simulink model "s_c_nbe_m1k"  (R2016b)
settings: Solver=VariableStepAuto  StartTime=0.0  StopTime=1000  RelTol=1e-3  EnableMultiTasking=on
undefined symbols (not defined in the file): Coeffs, fft_stages, n_taps, output_bits, pfb_coeff_gen_calc, xengbits
libraries: xbsIndex_r4 x23639, casper_library_misc x65, casper_library_scopes x4, xbsReplacements_r4 x4, xps_library x3
(part 19 of 198)

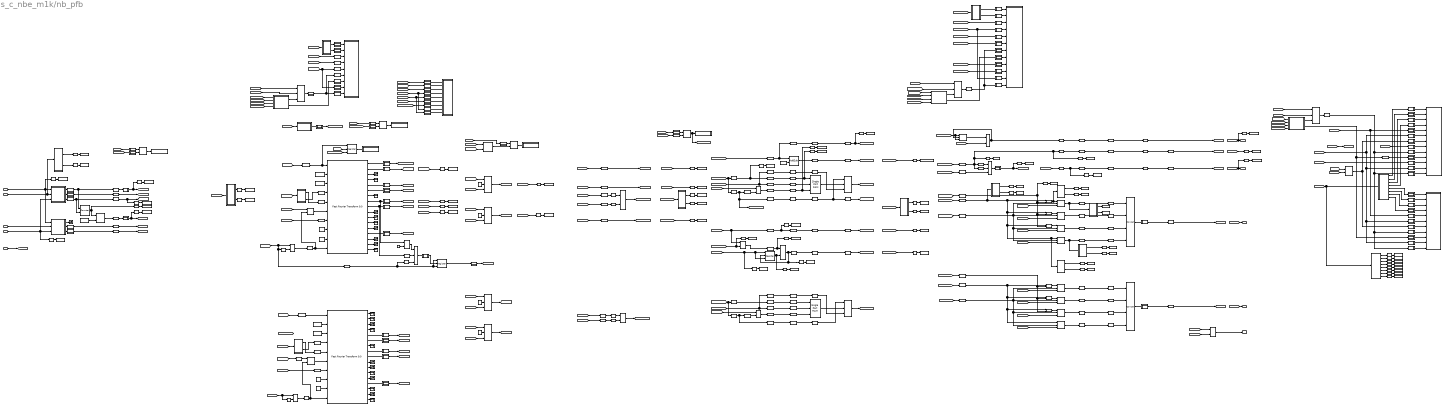
== system s_c_nbe_m1k/nb_pfb ==
  note: FWD = 1
  note: NOTE: Init script Disabled due to change to manual change to sync_delay block
  note: NOTE: The sync must be inline with the DV at this point
  note: Trigger sync on falling edge
  note: NOT ensures that a sync occuring atthe same time as ch=0 will prevent
      | sync from latching the register. The next cycle when sync in =0 the relational check
      | will equal 1  as the input will be zero as the FFT block would have just finished a reset.
  note: Only allow sync to occur when ch=0 and dv=1.
  note: Delay=2 as rst is 2 cycles. Prevents sync from popping out early
  note: Pass sync when first 4 samples have been captured
  note: Sanity check for channel number out
  note: Trigger when half the channels have been written
  note: Check if pol0 and pol1 ch outputs drift.
      | This should never happen.
  note: Needs to be 10b for 1k
  note: Count how many times the current_channel
      | is equal to 2^fft_stages BEFORE the sync occurs.
      | This is needed to compute the new time for the time gen
      | block which follows.
  note: There is no offset of the sync by 3 cycles. This is due to the 1:4
      | sample ratio casued by the capture_now. We want the sync to
      | occur one cycle before DV
  note: Wait for capture_now to trigger after sync has arrived
  note: Trigger capture_now every '4' samples.
      | This is based on the current channel index.
      | This starts at 0, so trigger when current channels
      | lower two bits = '1' and '1' (i.e. decimal 3).
  note: Needs to be 10b for 1k
  note: Trigger when half the channels have been written
  note: NOTE: The sync must be inline with the DV at this point
  note: FWD = 1
  sync : Inport
  pol0 : Inport  Port=2
  pol1 : Inport  Port=3
  dvalid : Inport  Port=4
  fft_shift : Inport  Port=5
  AddSub : xbsIndex_r4/AddSub  mode=Subtraction  use_carryin=off  use_carryout=off  en=off  latency=1  precision=User Defined  arith_type=Unsigned  n_bits=fft_stages-1  bin_pt=0  quantization=Truncate  overflow=Wrap  use_behavioral_HDL=off  hw_selection=Fabric  pipelined=off  dbl_ovrd=off  block_type=addsub
  Concat : xbsIndex_r4/Concat  num_inputs=2  dbl_ovrd=off  block_type=concat
  Concat1 : xbsIndex_r4/Concat  num_inputs=4  dbl_ovrd=off  block_type=concat
  Concat2 : xbsIndex_r4/Concat  num_inputs=2  dbl_ovrd=off  block_type=concat
  Concat3 : xbsIndex_r4/Concat  num_inputs=2  dbl_ovrd=off  block_type=concat
  Concat5 : xbsIndex_r4/Concat  num_inputs=4  dbl_ovrd=off  block_type=concat
  Constant : xbsIndex_r4/Constant  const=0  gui_display_data_type=Fixed-point  arith_type=Unsigned  n_bits=10  bin_pt=0  preci_type=Single  exp_width=8  frac_width=24  explicit_period=on  period=1  equ=P=C  opselect=C  inp2=PCIN>>17  opr=+  inp1=P  carry=CIN  dbl_ovrd=off  block_type=constant
  Constant{1..2,6..7} (4 alike) : xbsIndex_r4/Constant  const=0  gui_display_data_type=Fixed-point  arith_type=Signed (2's comp)  n_bits=18  bin_pt=17  preci_type=Single  exp_width=8  frac_width=24  explicit_period=on  period=1  equ=P=C  opselect=C  inp2=PCIN>>17  opr=+  inp1=P  carry=CIN  dbl_ovrd=off  block_type=constant
  Constant10 : xbsIndex_r4/Constant  const=1  gui_display_data_type=Boolean  arith_type=Boolean  n_bits=1  bin_pt=0  preci_type=Single  exp_width=8  frac_width=24  explicit_period=on  period=1  equ=P=C  opselect=C  inp2=PCIN>>17  opr=+  inp1=P  carry=CIN  dbl_ovrd=off  block_type=constant
  Constant{4,8,11..12} (4 alike) : xbsIndex_r4/Constant  const=1  gui_display_data_type=Boolean  arith_type=Boolean  n_bits=18  bin_pt=17  preci_type=Single  exp_width=8  frac_width=24  explicit_period=on  period=1  equ=P=C  opselect=C  inp2=PCIN>>17  opr=+  inp1=P  carry=CIN  dbl_ovrd=off  block_type=constant
  Constant13 : xbsIndex_r4/Constant  const=1  gui_display_data_type=Boolean  arith_type=Boolean  n_bits=1  bin_pt=0  preci_type=Single  exp_width=8  frac_width=24  explicit_period=on  period=1  equ=P=C  opselect=C  inp2=PCIN>>17  opr=+  inp1=P  carry=CIN  dbl_ovrd=off  block_type=constant
  Constant17 : xbsIndex_r4/Constant  const=2^(fft_stages-2)  gui_display_data_type=Fixed-point  arith_type=Unsigned  n_bits=fft_stages-1  bin_pt=0  preci_type=Single  exp_width=8  frac_width=24  explicit_period=on  period=1  equ=P=C  opselect=C  inp2=PCIN>>17  opr=+  inp1=P  carry=CIN  dbl_ovrd=off  block_type=constant
  Constant3 : xbsIndex_r4/Constant  const=1  gui_display_data_type=Fixed-point  arith_type=Unsigned  n_bits=1  bin_pt=0  preci_type=Single  exp_width=8  frac_width=24  explicit_period=on  period=1  equ=P=C  opselect=C  inp2=PCIN>>17  opr=+  inp1=P  carry=CIN  dbl_ovrd=off  block_type=constant
  Constant5 : xbsIndex_r4/Constant  const=1  gui_display_data_type=Fixed-point  arith_type=Unsigned  n_bits=1  bin_pt=0  preci_type=Single  exp_width=8  frac_width=24  explicit_period=on  period=1  equ=P=C  opselect=C  inp2=PCIN>>17  opr=+  inp1=P  carry=CIN  dbl_ovrd=off  block_type=constant
  Constant9 : xbsIndex_r4/Constant  const=(2^(fft_stages-1))-1  gui_display_data_type=Fixed-point  arith_type=Unsigned  n_bits=fft_stages+1  bin_pt=0  preci_type=Single  exp_width=8  frac_width=24  explicit_period=on  period=1  equ=P=C  opselect=C  inp2=PCIN>>17  opr=+  inp1=P  carry=CIN  dbl_ovrd=off  block_type=constant
  Counter1 : xbsIndex_r4/Counter  cnt_type=Free Running  cnt_to=Inf  operation=Up  start_count=0  cnt_by_val=1  arith_type=Unsigned  n_bits=4  bin_pt=0  load_pin=off  rst=on  en=on  explicit_period=on  period=1  use_behavioral_HDL=off  implementation=DSP48  dbl_ovrd=off  block_type=counter
  Counter12 : xbsIndex_r4/Counter  cnt_type=Free Running  cnt_to=Inf  operation=Up  start_count=0  cnt_by_val=1  arith_type=Unsigned  n_bits=32  bin_pt=0  load_pin=off  rst=on  en=on  explicit_period=on  period=1  use_behavioral_HDL=off  implementation=DSP48  dbl_ovrd=off  block_type=counter
      settings: block_version=11.4
  Counter2 : xbsIndex_r4/Counter  cnt_type=Free Running  cnt_to=Inf  operation=Up  start_count=0  cnt_by_val=1  arith_type=Unsigned  n_bits=32  bin_pt=0  load_pin=off  rst=on  en=on  explicit_period=on  period=1  use_behavioral_HDL=off  implementation=DSP48  dbl_ovrd=off  block_type=counter
      settings: block_version=11.4
  Counter3 : xbsIndex_r4/Counter  cnt_type=Free Running  cnt_to=Inf  operation=Up  start_count=0  cnt_by_val=1  arith_type=Unsigned  n_bits=fft_stages-1  bin_pt=0  load_pin=off  rst=on  en=on  explicit_period=on  period=1  use_behavioral_HDL=off  implementation=Fabric  dbl_ovrd=off  block_type=counter
  Counter4 : xbsIndex_r4/Counter  cnt_type=Free Running  cnt_to=Inf  operation=Up  start_count=0  cnt_by_val=1  arith_type=Unsigned  n_bits=11  bin_pt=0  load_pin=off  rst=on  en=on  explicit_period=on  period=1  use_behavioral_HDL=off  implementation=DSP48  dbl_ovrd=off  block_type=counter
      settings: block_version=11.4
  Counter5 : xbsIndex_r4/Counter  cnt_type=Free Running  cnt_to=Inf  operation=Up  start_count=0  cnt_by_val=1  arith_type=Unsigned  n_bits=8  bin_pt=0  load_pin=off  rst=on  en=on  explicit_period=on  period=1  use_behavioral_HDL=off  implementation=DSP48  dbl_ovrd=off  block_type=counter
      settings: block_version=11.4
  Delay{1..6,8..13,15,17..18,21..35,37..38,41..50,53..63,65,68,73..76,78,86..96,99..117} (90 alike) : xbsIndex_r4/Delay  rst=off  infoeditControl=Selection of Reset will increase slice count due to use of real FFs and instead of SRLs  en=off  latency=1  reg_retiming=off  dbl_ovrd=off  block_type=delay
      settings: infoedit=Hardware notes: A delay line is a chain, each link of which is an SRL16 or SRL32 followed by a flip-flop.
  Delay{14,39..40,67,69..70,81..84,118} (11 alike) : xbsIndex_r4/Delay  rst=off  infoeditControl=Selection of Reset will increase slice count due to use of real FFs and instead of SRLs  en=off  latency=2  reg_retiming=off  dbl_ovrd=off  block_type=delay
      settings: infoedit=Hardware notes: A delay line is a chain, each link of which is an SRL16 or SRL32 followed by a flip-flop.
  Delay16 : xbsIndex_r4/Delay  rst=off  infoeditControl=Selection of Reset will increase slice count due to use of real FFs and instead of SRLs  en=on  latency=3  reg_retiming=off  dbl_ovrd=off  block_type=delay
      settings: infoedit=Hardware notes: A delay line is a chain, each link of which is an SRL16 or SRL32 followed by a flip-flop.
  Delay19 : xbsIndex_r4/Delay  rst=off  infoeditControl=Selection of Reset will increase slice count due to use of real FFs and instead of SRLs  en=on  latency=2  reg_retiming=off  dbl_ovrd=off  block_type=delay
      settings: infoedit=Hardware notes: A delay line is a chain, each link of which is an SRL16 or SRL32 followed by a flip-flop.
  Delay20 : xbsIndex_r4/Delay  rst=off  infoeditControl=Selection of Reset will increase slice count due to use of real FFs and instead of SRLs  en=on  latency=1  reg_retiming=off  dbl_ovrd=off  block_type=delay
      settings: infoedit=Hardware notes: A delay line is a chain, each link of which is an SRL16 or SRL32 followed by a flip-flop.
  Delay51 : xbsIndex_r4/Delay  rst=off  infoeditControl=Selection of Reset will increase slice count due to use of real FFs and instead of SRLs  en=on  latency=2  reg_retiming=off  dbl_ovrd=off  block_type=delay
      settings: infoedit=Hardware notes: A delay line is a chain, each link of which is an SRL16 or SRL32 followed by a flip-flop.
  Delay52 : xbsIndex_r4/Delay  rst=off  infoeditControl=Selection of Reset will increase slice count due to use of real FFs and instead of SRLs  en=on  latency=1  reg_retiming=off  dbl_ovrd=off  block_type=delay
      settings: infoedit=Hardware notes: A delay line is a chain, each link of which is an SRL16 or SRL32 followed by a flip-flop.
  Delay7 : xbsIndex_r4/Delay  rst=off  infoeditControl=Selection of Reset will increase slice count due to use of real FFs and instead of SRLs  en=on  latency=3  reg_retiming=off  dbl_ovrd=off  block_type=delay
      settings: infoedit=Hardware notes: A delay line is a chain, each link of which is an SRL16 or SRL32 followed by a flip-flop.
  Delay97 : xbsIndex_r4/Delay  rst=off  infoeditControl=Selection of Reset will increase slice count due to use of real FFs and instead of SRLs  en=off  latency=1  reg_retiming=on  dbl_ovrd=off  block_type=delay
  Delay98 : xbsIndex_r4/Delay  rst=off  infoeditControl=Selection of Reset will increase slice count due to use of real FFs and instead of SRLs  en=off  latency=1  reg_retiming=on  dbl_ovrd=off  block_type=delay
  Fast Fourier Transform 9.0 1 : xbsIndex_r4/Fast Fourier Transform 9.0   transform_length=1024  target_clock_frequency=240  target_data_throughput=50  implementation_options=pipelined_streaming_io  run_time_configurable_transform_length=off  phase_factor_width=18  scaling_options=scaled  rounding_modes=convergent_rounding  aclken=off  aresetn=on  output_ordering=natural_order  cyclic_prefix_insertion=off  throttle_scheme=nonrealtime  xk_index=on  ovflo=on  trim_axipin_name=on  memory_options_data=block_ram  memory_options_phase_factors=block_ram  number_of_stages_using_block_ram_for_data_and_phase_factors=5  memory_options_reorder=block_ram  memory_options_hybrid=off  complex_mult_type=use_mults_performance  butterfly_type=use_xtremedsp_slices  simulation_type=hybrid_sim  simulation_model=sysgen:xfftv9_cmodel  data_path_portlist={ 's_axis_data_tdata', 'm_axis_data_tdata', 'm_axis_status_tdata', 'event_fft_overflow' }  channels=1  input_ordering=natural_order  input_width=16  ip_name=Fast Fourier Transform  ip_version=9.0  dsptool_ready=true  ipcore_usecache=true  ipcore_useipmodelcache=true  wrapper_available=true  port_translation_map={ 'aclken' => 'en', 'aresetn' => 'rst'}  data_format=fixed_point  block_type=xfft_v9_0
  Fast Fourier Transform 9.0 2 : xbsIndex_r4/Fast Fourier Transform 9.0   transform_length=1024  target_clock_frequency=240  target_data_throughput=50  implementation_options=pipelined_streaming_io  run_time_configurable_transform_length=off  phase_factor_width=18  scaling_options=scaled  rounding_modes=convergent_rounding  aclken=off  aresetn=on  output_ordering=natural_order  cyclic_prefix_insertion=off  throttle_scheme=nonrealtime  xk_index=on  ovflo=on  trim_axipin_name=on  memory_options_data=block_ram  memory_options_phase_factors=block_ram  number_of_stages_using_block_ram_for_data_and_phase_factors=5  memory_options_reorder=block_ram  memory_options_hybrid=off  complex_mult_type=use_mults_performance  butterfly_type=use_xtremedsp_slices  simulation_type=hybrid_sim  simulation_model=sysgen:xfftv9_cmodel  data_path_portlist={ 's_axis_data_tdata', 'm_axis_data_tdata', 'm_axis_status_tdata', 'event_fft_overflow' }  channels=1  input_ordering=natural_order  input_width=16  ip_name=Fast Fourier Transform  ip_version=9.0  dsptool_ready=true  ipcore_usecache=true  ipcore_useipmodelcache=true  wrapper_available=true  port_translation_map={ 'aclken' => 'en', 'aresetn' => 'rst'}  data_format=fixed_point  block_type=xfft_v9_0
  Gateway Out{1..9,11..31,33..40,43,46..53,55..58,61,65..67,70..73,83} (60 alike) : xbsIndex_r4/Gateway Out  inherit_from_input=off  hdl_port=on  rows=1  columns=1  UseAsDAC=off  DACChannel='1'  interface=None  automatic_assignment=on  address_offset=hex2dec('00')  intf_name=''  intf_description=''  timing_constraint=None  locs_specified=off  LOCs={}  io_standard={}  block_type=gatewayout
  Inverter{,1..4} (5 alike) : xbsIndex_r4/Inverter  en=off  latency=0  dbl_ovrd=off  block_type=inv
  Logical : xbsIndex_r4/Logical  logical_function=AND  inputs=3  en=off  latency=0  precision=Full  arith_type=Unsigned  n_bits=16  bin_pt=0  align_bp=on  dbl_ovrd=off  block_type=logical
  Logical{1..3,5..6,8,10} (7 alike) : xbsIndex_r4/Logical  logical_function=AND  inputs=2  en=off  latency=0  precision=Full  arith_type=Unsigned  n_bits=16  bin_pt=0  align_bp=on  dbl_ovrd=off  block_type=logical
  Logical11 : xbsIndex_r4/Logical  logical_function=OR  inputs=2  en=off  latency=0  precision=Full  arith_type=Unsigned  n_bits=16  bin_pt=0  align_bp=on  dbl_ovrd=off  block_type=logical
  Logical4 : xbsIndex_r4/Logical  logical_function=AND  inputs=3  en=off  latency=0  precision=Full  arith_type=Unsigned  n_bits=16  bin_pt=0  align_bp=on  dbl_ovrd=off  block_type=logical
  Logical7 : xbsIndex_r4/Logical  logical_function=OR  inputs=2  en=off  latency=0  precision=Full  arith_type=Unsigned  n_bits=16  bin_pt=0  align_bp=on  dbl_ovrd=off  block_type=logical
  Mux1 : xbsIndex_r4/Mux  inputs=2  en=off  latency=1  precision=Full  arith_type=Unsigned  n_bits=16  bin_pt=14  quantization=Truncate  overflow=Wrap  dbl_ovrd=off  block_type=mux
  Mux{3..6,8..10} (7 alike) : xbsIndex_r4/Mux  inputs=2  en=off  latency=0  precision=Full  arith_type=Unsigned  n_bits=16  bin_pt=14  quantization=Truncate  overflow=Wrap  dbl_ovrd=off  block_type=mux
  Mux11 : xbsIndex_r4/Mux  inputs=2  en=off  latency=1  precision=Full  arith_type=Unsigned  n_bits=16  bin_pt=14  quantization=Truncate  overflow=Wrap  dbl_ovrd=off  block_type=mux
  Register{,1..7,9..12} (12 alike) : xbsIndex_r4/Register  init=0  rst=on  en=on  dbl_ovrd=off  block_type=register
  Reinterpret{,1..3} (4 alike) : xbsIndex_r4/Reinterpret  force_arith_type=on  arith_type=Unsigned  force_bin_pt=on  bin_pt=0  block_type=reinterpret
  Relational1 : xbsIndex_r4/Relational  mode=a!=b  op_type=Bool  en=off  latency=4  dbl_ovrd=off  block_type=relational
  Relational2 : xbsIndex_r4/Relational  mode=a=b  op_type=Bool  en=off  latency=1  dbl_ovrd=off  block_type=relational
  Relational4 : xbsIndex_r4/Relational  mode=a=b  op_type=Bool  en=off  latency=1  dbl_ovrd=off  block_type=relational
  Single Port RAM : xbsIndex_r4/Single Port RAM  depth=2^(fft_stages-2)  initVector=0  distributed_mem=Block RAM  write_mode=Read Before Write  rst=off  init_reg=0  en=off  latency=1  optimize=Area  dbl_ovrd=off  block_type=spram
  Single Port RAM1 : xbsIndex_r4/Single Port RAM  depth=2^(fft_stages-2)  initVector=0  distributed_mem=Block RAM  write_mode=Read Before Write  rst=off  init_reg=0  en=off  latency=1  optimize=Area  dbl_ovrd=off  block_type=spram
  Slice : xbsIndex_r4/Slice  nbits=10  boolean_output=off  mode=Lower Bit Location + Width  bit1=0  base1=MSB of Input  bit0=0  base0=LSB of Input  dbl_ovrd=off  block_type=slice
  Slice1 : xbsIndex_r4/Slice  nbits=10  boolean_output=off  mode=Lower Bit Location + Width  bit1=0  base1=MSB of Input  bit0=0  base0=LSB of Input  dbl_ovrd=off  block_type=slice
  Slice2 : xbsIndex_r4/Slice  nbits=1  boolean_output=on  mode=Lower Bit Location + Width  bit1=0  base1=MSB of Input  bit0=fft_stages-2  base0=LSB of Input  dbl_ovrd=off  block_type=slice
  Slice3 : xbsIndex_r4/Slice  nbits=1  boolean_output=on  mode=Lower Bit Location + Width  bit1=0  base1=MSB of Input  bit0=fft_stages-2  base0=LSB of Input  dbl_ovrd=off  block_type=slice
  Slice4 : xbsIndex_r4/Slice  nbits=fft_stages-2  boolean_output=off  mode=Lower Bit Location + Width  bit1=0  base1=MSB of Input  bit0=0  base0=LSB of Input  dbl_ovrd=off  block_type=slice
  Slice5 : xbsIndex_r4/Slice  nbits=38  boolean_output=off  mode=Lower Bit Location + Width  bit1=0  base1=MSB of Input  bit0=0  base0=LSB of Input  dbl_ovrd=off  block_type=slice
  Slice6 : xbsIndex_r4/Slice  nbits=fft_stages-2  boolean_output=off  mode=Lower Bit Location + Width  bit1=0  base1=MSB of Input  bit0=0  base0=LSB of Input  dbl_ovrd=off  block_type=slice
  Terminator{1..5,7..24} (23 alike) : Terminator
  To Workspace1 : ToWorkspace  VariableName=fir_dv  SaveFormat=Timeseries  SampleTime=-1
  To Workspace11 : ToWorkspace  VariableName=fft_ch_out1  SaveFormat=Timeseries  SampleTime=-1
  To Workspace12 : ToWorkspace  VariableName=cap_tp6  SaveFormat=Timeseries  SampleTime=-1
  To Workspace13 : ToWorkspace  VariableName=cap_tp7  SaveFormat=Timeseries  SampleTime=-1
  To Workspace14 : ToWorkspace  VariableName=cap_tp8  SaveFormat=Timeseries  SampleTime=-1
  To Workspace15 : ToWorkspace  VariableName=fft_re1  SaveFormat=Timeseries  SampleTime=-1
  To Workspace16 : ToWorkspace  VariableName=fft_sync  SaveFormat=Timeseries  SampleTime=-1
  To Workspace17 : ToWorkspace  VariableName=fft_im1  SaveFormat=Timeseries  SampleTime=-1
  To Workspace18 : ToWorkspace  VariableName=fft_tp1  SaveFormat=Timeseries  SampleTime=-1
  To Workspace19 : ToWorkspace  VariableName=nb_dv  SaveFormat=Timeseries  SampleTime=-1
  To Workspace2 : ToWorkspace  VariableName=fft_re  SaveFormat=Timeseries  SampleTime=-1
  To Workspace20 : ToWorkspace  VariableName=fft_tp  SaveFormat=Timeseries  SampleTime=-1
  To Workspace21 : ToWorkspace  VariableName=nb_r0  SaveFormat=Timeseries  SampleTime=-1
  To Workspace22 : ToWorkspace  VariableName=cap_tp21  SaveFormat=Timeseries  SampleTime=-1
  To Workspace23 : ToWorkspace  VariableName=nb_i0  SaveFormat=Timeseries  SampleTime=-1
  To Workspace24 : ToWorkspace  VariableName=nb_r1  SaveFormat=Timeseries  SampleTime=-1
  To Workspace25 : ToWorkspace  VariableName=nb_r2  SaveFormat=Timeseries  SampleTime=-1
  To Workspace26 : ToWorkspace  VariableName=nb_r3  SaveFormat=Timeseries  SampleTime=-1
  To Workspace27 : ToWorkspace  VariableName=nb_i1  SaveFormat=Timeseries  SampleTime=-1
  To Workspace28 : ToWorkspace  VariableName=nb_i2  SaveFormat=Timeseries  SampleTime=-1
  To Workspace29 : ToWorkspace  VariableName=nb_i3  SaveFormat=Timeseries  SampleTime=-1
  To Workspace3 : ToWorkspace  VariableName=fft_dvalid  SaveFormat=Timeseries  SampleTime=-1
  To Workspace30 : ToWorkspace  VariableName=cap_tp22  SaveFormat=Timeseries  SampleTime=-1
  To Workspace31 : ToWorkspace  VariableName=fft_tp2  SaveFormat=Timeseries  SampleTime=-1
  To Workspace32 : ToWorkspace  VariableName=fft_ch  SaveFormat=Timeseries  SampleTime=-1
  To Workspace34 : ToWorkspace  VariableName=fft_tp3  SaveFormat=Timeseries  SampleTime=-1
  To Workspace35 : ToWorkspace  VariableName=fir_p1  SaveFormat=Timeseries  SampleTime=-1
  To Workspace36 : ToWorkspace  VariableName=fir_dv1  SaveFormat=Timeseries  SampleTime=-1
  To Workspace37 : ToWorkspace  VariableName=fft_sync0  SaveFormat=Timeseries  SampleTime=-1
  To Workspace38 : ToWorkspace  VariableName=cap_tp23  SaveFormat=Timeseries  SampleTime=-1
  To Workspace39 : ToWorkspace  VariableName=fir_p  SaveFormat=Timeseries  SampleTime=-1
  To Workspace4 : ToWorkspace  VariableName=fir_re  SaveFormat=Timeseries  SampleTime=-1
  To Workspace40 : ToWorkspace  VariableName=capture_now  SaveFormat=Timeseries  SampleTime=-1
  To Workspace42 : ToWorkspace  VariableName=reord_sync  SaveFormat=Timeseries  SampleTime=-1
  To Workspace43 : ToWorkspace  VariableName=fft_tp4  SaveFormat=Timeseries  SampleTime=-1
  To Workspace45 : ToWorkspace  VariableName=cap_tp9  SaveFormat=Timeseries  SampleTime=-1
  To Workspace46 : ToWorkspace  VariableName=cap_tp10  SaveFormat=Timeseries  SampleTime=-1
  To Workspace47 : ToWorkspace  VariableName=reord_dv  SaveFormat=Timeseries  SampleTime=-1
  To Workspace48 : ToWorkspace  VariableName=fft_tp5  SaveFormat=Timeseries  SampleTime=-1
  To Workspace49 : ToWorkspace  VariableName=nb_dv1  SaveFormat=Timeseries  SampleTime=-1
  To Workspace5 : ToWorkspace  VariableName=fft_im  SaveFormat=Timeseries  SampleTime=-1
  To Workspace51 : ToWorkspace  VariableName=reord_ch  SaveFormat=Timeseries  SampleTime=-1
  To Workspace53 : ToWorkspace  VariableName=fir_tlast  SaveFormat=Timeseries  SampleTime=-1
  To Workspace54 : ToWorkspace  VariableName=fir_tlast1  SaveFormat=Timeseries  SampleTime=-1
  To Workspace56 : ToWorkspace  VariableName=fft_tp6  SaveFormat=Timeseries  SampleTime=-1
  To Workspace57 : ToWorkspace  VariableName=fft_tp7  SaveFormat=Timeseries  SampleTime=-1
  To Workspace58 : ToWorkspace  VariableName=fft_ch_reord  SaveFormat=Timeseries  SampleTime=-1
  To Workspace59 : ToWorkspace  VariableName=fft_tp8  SaveFormat=Timeseries  SampleTime=-1
  To Workspace6 : ToWorkspace  VariableName=fir_sync  SaveFormat=Timeseries  SampleTime=-1
  To Workspace64 : ToWorkspace  VariableName=cap_tp11  SaveFormat=Timeseries  SampleTime=-1
  To Workspace65 : ToWorkspace  VariableName=fft_ch0  SaveFormat=Timeseries  SampleTime=-1
  To Workspace66 : ToWorkspace  VariableName=fft_dv0  SaveFormat=Timeseries  SampleTime=-1
  To Workspace69 : ToWorkspace  VariableName=fft_re2  SaveFormat=Timeseries  SampleTime=-1
  To Workspace7 : ToWorkspace  VariableName=nb_sync  SaveFormat=Timeseries  SampleTime=-1
  To Workspace70 : ToWorkspace  VariableName=fft_im2  SaveFormat=Timeseries  SampleTime=-1
  To Workspace71 : ToWorkspace  VariableName=fft_tready0  SaveFormat=Timeseries  SampleTime=-1
  To Workspace73 : ToWorkspace  VariableName=cap_tp12  SaveFormat=Timeseries  SampleTime=-1
  To Workspace74 : ToWorkspace  VariableName=cap_tp13  SaveFormat=Timeseries  SampleTime=-1
  To Workspace75 : ToWorkspace  VariableName=cap_tp14  SaveFormat=Timeseries  SampleTime=-1
  To Workspace8 : ToWorkspace  VariableName=fir_im  SaveFormat=Timeseries  SampleTime=-1
  To Workspace85 : ToWorkspace  VariableName=fft_ch_out  SaveFormat=Timeseries  SampleTime=-1
  To Workspace9 : ToWorkspace  VariableName=fir_sync1  SaveFormat=Timeseries  SampleTime=-1
  bus_expand1 : Subsystem  AncestorBlock=casper_library_flow_control/bus_expand  mask(bus_expand){mode=divisions of equal size, outputNum=8, outputWidth=18, outputBinaryPt=17, outputArithmeticType=1, show_format=off, outputToWorkspace=off, variablePrefix=out, outputToModelAsWell=on}
      mask prompts: outputNum "Number of outputs:"; outputWidth "Output width:"; outputBinaryPt "Output binary point position:"; outputArithmeticType "Output arithmetic type (ufix=0, fix=1, bool=2):"; show_format "Print format string?"; outputToWorkspace "Output to workspace?"; variablePrefix "Variable name prefix:"; outputToModelAsWell "Output to model as well?"
      mask help:
      | Expands a 'bus' made using a bus_create or Xilinx
      | concat block.
      | The input will be divided into the specified number
      | of outputs with the specified arithmetic types.
      | Divisions are made from most significant bit.
      mask init: same as s_c_nbe_m1k/bus_expand1
      settings: AttributesFormatString=8 outputs
      mask TypeOptions mode: divisions of equal size | divisions of arbitrary size
      mask Callback mode: bus_expand_callback();
      mask Callback outputWidth: bus_expand_callback();
      mask Callback outputToWorkspace: bus_expand_callback();
  bus_expand10 : Subsystem  AncestorBlock=casper_library_flow_control/bus_expand  mask(bus_expand){mode=divisions of equal size, outputNum=2, outputWidth=18, outputBinaryPt=17, outputArithmeticType=1, show_format=off, outputToWorkspace=off, variablePrefix=out, outputToModelAsWell=on}
      mask prompts: outputNum "Number of outputs:"; outputWidth "Output width:"; outputBinaryPt "Output binary point position:"; outputArithmeticType "Output arithmetic type (ufix=0, fix=1, bool=2):"; show_format "Print format string?"; outputToWorkspace "Output to workspace?"; variablePrefix "Variable name prefix:"; outputToModelAsWell "Output to model as well?"
      mask help:
      | Expands a 'bus' made using a bus_create or Xilinx
      | concat block.
      | The input will be divided into the specified number
      | of outputs with the specified arithmetic types.
      | Divisions are made from most significant bit.
      mask init: same as s_c_nbe_m1k/bus_expand1
      settings: AttributesFormatString=2 outputs
      mask TypeOptions mode: divisions of equal size | divisions of arbitrary size
      mask Callback mode: bus_expand_callback();
      mask Callback outputWidth: bus_expand_callback();
      mask Callback outputToWorkspace: bus_expand_callback();
  bus_expand11 : Subsystem  AncestorBlock=casper_library_flow_control/bus_expand  mask(bus_expand){mode=divisions of equal size, outputNum=2, outputWidth=18, outputBinaryPt=17, outputArithmeticType=1, show_format=off, outputToWorkspace=off, variablePrefix=out, outputToModelAsWell=on}
      mask prompts: outputNum "Number of outputs:"; outputWidth "Output width:"; outputBinaryPt "Output binary point position:"; outputArithmeticType "Output arithmetic type (ufix=0, fix=1, bool=2):"; show_format "Print format string?"; outputToWorkspace "Output to workspace?"; variablePrefix "Variable name prefix:"; outputToModelAsWell "Output to model as well?"
      mask help:
      | Expands a 'bus' made using a bus_create or Xilinx
      | concat block.
      | The input will be divided into the specified number
      | of outputs with the specified arithmetic types.
      | Divisions are made from most significant bit.
      mask init: same as s_c_nbe_m1k/bus_expand1
      settings: AttributesFormatString=2 outputs
      mask TypeOptions mode: divisions of equal size | divisions of arbitrary size
      mask Callback mode: bus_expand_callback();
      mask Callback outputWidth: bus_expand_callback();
      mask Callback outputToWorkspace: bus_expand_callback();
  bus_expand12 : Subsystem  AncestorBlock=casper_library_flow_control/bus_expand  mask(bus_expand){mode=divisions of equal size, outputNum=2, outputWidth=18, outputBinaryPt=17, outputArithmeticType=1, show_format=off, outputToWorkspace=off, variablePrefix=out, outputToModelAsWell=on}
      mask prompts: outputNum "Number of outputs:"; outputWidth "Output width:"; outputBinaryPt "Output binary point position:"; outputArithmeticType "Output arithmetic type (ufix=0, fix=1, bool=2):"; show_format "Print format string?"; outputToWorkspace "Output to workspace?"; variablePrefix "Variable name prefix:"; outputToModelAsWell "Output to model as well?"
      mask help:
      | Expands a 'bus' made using a bus_create or Xilinx
      | concat block.
      | The input will be divided into the specified number
      | of outputs with the specified arithmetic types.
      | Divisions are made from most significant bit.
      mask init: same as s_c_nbe_m1k/bus_expand1
      settings: AttributesFormatString=2 outputs
      mask TypeOptions mode: divisions of equal size | divisions of arbitrary size
      mask Callback mode: bus_expand_callback();
      mask Callback outputWidth: bus_expand_callback();
      mask Callback outputToWorkspace: bus_expand_callback();
  bus_expand13 : Subsystem  AncestorBlock=casper_library_flow_control/bus_expand  mask(bus_expand){mode=divisions of equal size, outputNum=2, outputWidth=18, outputBinaryPt=17, outputArithmeticType=1, show_format=off, outputToWorkspace=off, variablePrefix=out, outputToModelAsWell=on}
      mask prompts: outputNum "Number of outputs:"; outputWidth "Output width:"; outputBinaryPt "Output binary point position:"; outputArithmeticType "Output arithmetic type (ufix=0, fix=1, bool=2):"; show_format "Print format string?"; outputToWorkspace "Output to workspace?"; variablePrefix "Variable name prefix:"; outputToModelAsWell "Output to model as well?"
      mask help:
      | Expands a 'bus' made using a bus_create or Xilinx
      | concat block.
      | The input will be divided into the specified number
      | of outputs with the specified arithmetic types.
      | Divisions are made from most significant bit.
      mask init: same as s_c_nbe_m1k/bus_expand1
      settings: AttributesFormatString=2 outputs
      mask TypeOptions mode: divisions of equal size | divisions of arbitrary size
      mask Callback mode: bus_expand_callback();
      mask Callback outputWidth: bus_expand_callback();
      mask Callback outputToWorkspace: bus_expand_callback();
  bus_expand14 : Subsystem  AncestorBlock=casper_library_flow_control/bus_expand  mask(bus_expand){mode=divisions of equal size, outputNum=2, outputWidth=10, outputBinaryPt=9, outputArithmeticType=1, show_format=off, outputToWorkspace=off, variablePrefix=out, outputToModelAsWell=on}
      mask prompts: outputNum "Number of outputs:"; outputWidth "Output width:"; outputBinaryPt "Output binary point position:"; outputArithmeticType "Output arithmetic type (ufix=0, fix=1, bool=2):"; show_format "Print format string?"; outputToWorkspace "Output to workspace?"; variablePrefix "Variable name prefix:"; outputToModelAsWell "Output to model as well?"
      mask help:
      | Expands a 'bus' made using a bus_create or Xilinx
      | concat block.
      | The input will be divided into the specified number
      | of outputs with the specified arithmetic types.
      | Divisions are made from most significant bit.
      mask init: same as s_c_nbe_m1k/bus_expand1
      settings: AttributesFormatString=2 outputs
      mask TypeOptions mode: divisions of equal size | divisions of arbitrary size
      mask Callback mode: bus_expand_callback();
      mask Callback outputWidth: bus_expand_callback();
      mask Callback outputToWorkspace: bus_expand_callback();
  bus_expand16 : Subsystem  AncestorBlock=casper_library_flow_control/bus_expand  mask(bus_expand){mode=divisions of equal size, outputNum=2, outputWidth=18, outputBinaryPt=17, outputArithmeticType=1, show_format=off, outputToWorkspace=off, variablePrefix=out, outputToModelAsWell=on}
      mask prompts: outputNum "Number of outputs:"; outputWidth "Output width:"; outputBinaryPt "Output binary point position:"; outputArithmeticType "Output arithmetic type (ufix=0, fix=1, bool=2):"; show_format "Print format string?"; outputToWorkspace "Output to workspace?"; variablePrefix "Variable name prefix:"; outputToModelAsWell "Output to model as well?"
      mask help:
      | Expands a 'bus' made using a bus_create or Xilinx
      | concat block.
      | The input will be divided into the specified number
      | of outputs with the specified arithmetic types.
      | Divisions are made from most significant bit.
      mask init: same as s_c_nbe_m1k/bus_expand1
      settings: AttributesFormatString=2 outputs
      mask TypeOptions mode: divisions of equal size | divisions of arbitrary size
      mask Callback mode: bus_expand_callback();
      mask Callback outputWidth: bus_expand_callback();
      mask Callback outputToWorkspace: bus_expand_callback();
  bus_expand2 : Subsystem  AncestorBlock=casper_library_flow_control/bus_expand  mask(bus_expand){mode=divisions of equal size, outputNum=8, outputWidth=18, outputBinaryPt=17, outputArithmeticType=1, show_format=off, outputToWorkspace=off, variablePrefix=out, outputToModelAsWell=on}
      mask prompts: outputNum "Number of outputs:"; outputWidth "Output width:"; outputBinaryPt "Output binary point position:"; outputArithmeticType "Output arithmetic type (ufix=0, fix=1, bool=2):"; show_format "Print format string?"; outputToWorkspace "Output to workspace?"; variablePrefix "Variable name prefix:"; outputToModelAsWell "Output to model as well?"
      mask help:
      | Expands a 'bus' made using a bus_create or Xilinx
      | concat block.
      | The input will be divided into the specified number
      | of outputs with the specified arithmetic types.
      | Divisions are made from most significant bit.
      mask init: same as s_c_nbe_m1k/bus_expand1
      settings: AttributesFormatString=8 outputs
      mask TypeOptions mode: divisions of equal size | divisions of arbitrary size
      mask Callback mode: bus_expand_callback();
      mask Callback outputWidth: bus_expand_callback();
      mask Callback outputToWorkspace: bus_expand_callback();
  bus_expand3 : Subsystem  AncestorBlock=casper_library_flow_control/bus_expand  mask(bus_expand){mode=divisions of equal size, outputNum=2, outputWidth=18, outputBinaryPt=17, outputArithmeticType=1, show_format=off, outputToWorkspace=off, variablePrefix=out, outputToModelAsWell=on}
      mask prompts: outputNum "Number of outputs:"; outputWidth "Output width:"; outputBinaryPt "Output binary point position:"; outputArithmeticType "Output arithmetic type (ufix=0, fix=1, bool=2):"; show_format "Print format string?"; outputToWorkspace "Output to workspace?"; variablePrefix "Variable name prefix:"; outputToModelAsWell "Output to model as well?"
      mask help:
      | Expands a 'bus' made using a bus_create or Xilinx
      | concat block.
      | The input will be divided into the specified number
      | of outputs with the specified arithmetic types.
      | Divisions are made from most significant bit.
      mask init: same as s_c_nbe_m1k/bus_expand1
      settings: AttributesFormatString=2 outputs
      mask TypeOptions mode: divisions of equal size | divisions of arbitrary size
      mask Callback mode: bus_expand_callback();
      mask Callback outputWidth: bus_expand_callback();
      mask Callback outputToWorkspace: bus_expand_callback();
  bus_expand4 : Subsystem  AncestorBlock=casper_library_flow_control/bus_expand  mask(bus_expand){mode=divisions of equal size, outputNum=2, outputWidth=18, outputBinaryPt=17, outputArithmeticType=1, show_format=off, outputToWorkspace=off, variablePrefix=out, outputToModelAsWell=on}
      mask prompts: outputNum "Number of outputs:"; outputWidth "Output width:"; outputBinaryPt "Output binary point position:"; outputArithmeticType "Output arithmetic type (ufix=0, fix=1, bool=2):"; show_format "Print format string?"; outputToWorkspace "Output to workspace?"; variablePrefix "Variable name prefix:"; outputToModelAsWell "Output to model as well?"
      mask help:
      | Expands a 'bus' made using a bus_create or Xilinx
      | concat block.
      | The input will be divided into the specified number
      | of outputs with the specified arithmetic types.
      | Divisions are made from most significant bit.
      mask init: same as s_c_nbe_m1k/bus_expand1
      settings: AttributesFormatString=2 outputs
      mask TypeOptions mode: divisions of equal size | divisions of arbitrary size
      mask Callback mode: bus_expand_callback();
      mask Callback outputWidth: bus_expand_callback();
      mask Callback outputToWorkspace: bus_expand_callback();
  bus_expand5 : Subsystem  AncestorBlock=casper_library_flow_control/bus_expand  mask(bus_expand){mode=divisions of equal size, outputNum=2, outputWidth=18, outputBinaryPt=17, outputArithmeticType=1, show_format=off, outputToWorkspace=off, variablePrefix=out, outputToModelAsWell=on}
      mask prompts: outputNum "Number of outputs:"; outputWidth "Output width:"; outputBinaryPt "Output binary point position:"; outputArithmeticType "Output arithmetic type (ufix=0, fix=1, bool=2):"; show_format "Print format string?"; outputToWorkspace "Output to workspace?"; variablePrefix "Variable name prefix:"; outputToModelAsWell "Output to model as well?"
      mask help:
      | Expands a 'bus' made using a bus_create or Xilinx
      | concat block.
      | The input will be divided into the specified number
      | of outputs with the specified arithmetic types.
      | Divisions are made from most significant bit.
      mask init: same as s_c_nbe_m1k/bus_expand1
      settings: AttributesFormatString=2 outputs
      mask TypeOptions mode: divisions of equal size | divisions of arbitrary size
      mask Callback mode: bus_expand_callback();
      mask Callback outputWidth: bus_expand_callback();
      mask Callback outputToWorkspace: bus_expand_callback();
  bus_expand6 : Subsystem  AncestorBlock=casper_library_flow_control/bus_expand  mask(bus_expand){mode=divisions of equal size, outputNum=2, outputWidth=18, outputBinaryPt=17, outputArithmeticType=1, show_format=off, outputToWorkspace=off, variablePrefix=out, outputToModelAsWell=on}
      mask prompts: outputNum "Number of outputs:"; outputWidth "Output width:"; outputBinaryPt "Output binary point position:"; outputArithmeticType "Output arithmetic type (ufix=0, fix=1, bool=2):"; show_format "Print format string?"; outputToWorkspace "Output to workspace?"; variablePrefix "Variable name prefix:"; outputToModelAsWell "Output to model as well?"
      mask help:
      | Expands a 'bus' made using a bus_create or Xilinx
      | concat block.
      | The input will be divided into the specified number
      | of outputs with the specified arithmetic types.
      | Divisions are made from most significant bit.
      mask init: same as s_c_nbe_m1k/bus_expand1
      settings: AttributesFormatString=2 outputs
      mask TypeOptions mode: divisions of equal size | divisions of arbitrary size
      mask Callback mode: bus_expand_callback();
      mask Callback outputWidth: bus_expand_callback();
      mask Callback outputToWorkspace: bus_expand_callback();
  bus_expand7 : Subsystem  AncestorBlock=casper_library_flow_control/bus_expand  mask(bus_expand){mode=divisions of equal size, outputNum=2, outputWidth=18, outputBinaryPt=17, outputArithmeticType=1, show_format=off, outputToWorkspace=off, variablePrefix=out, outputToModelAsWell=on}
      mask prompts: outputNum "Number of outputs:"; outputWidth "Output width:"; outputBinaryPt "Output binary point position:"; outputArithmeticType "Output arithmetic type (ufix=0, fix=1, bool=2):"; show_format "Print format string?"; outputToWorkspace "Output to workspace?"; variablePrefix "Variable name prefix:"; outputToModelAsWell "Output to model as well?"
      mask help:
      | Expands a 'bus' made using a bus_create or Xilinx
      | concat block.
      | The input will be divided into the specified number
      | of outputs with the specified arithmetic types.
      | Divisions are made from most significant bit.
      mask init: same as s_c_nbe_m1k/bus_expand1
      settings: AttributesFormatString=2 outputs
      mask TypeOptions mode: divisions of equal size | divisions of arbitrary size
      mask Callback mode: bus_expand_callback();
      mask Callback outputWidth: bus_expand_callback();
      mask Callback outputToWorkspace: bus_expand_callback();
  bus_expand8 : Subsystem  AncestorBlock=casper_library_flow_control/bus_expand  mask(bus_expand){mode=divisions of equal size, outputNum=2, outputWidth=18, outputBinaryPt=17, outputArithmeticType=1, show_format=off, outputToWorkspace=off, variablePrefix=out, outputToModelAsWell=on}
      mask prompts: outputNum "Number of outputs:"; outputWidth "Output width:"; outputBinaryPt "Output binary point position:"; outputArithmeticType "Output arithmetic type (ufix=0, fix=1, bool=2):"; show_format "Print format string?"; outputToWorkspace "Output to workspace?"; variablePrefix "Variable name prefix:"; outputToModelAsWell "Output to model as well?"
      mask help:
      | Expands a 'bus' made using a bus_create or Xilinx
      | concat block.
      | The input will be divided into the specified number
      | of outputs with the specified arithmetic types.
      | Divisions are made from most significant bit.
      mask init: same as s_c_nbe_m1k/bus_expand1
      settings: AttributesFormatString=2 outputs
      mask TypeOptions mode: divisions of equal size | divisions of arbitrary size
      mask Callback mode: bus_expand_callback();
      mask Callback outputWidth: bus_expand_callback();
      mask Callback outputToWorkspace: bus_expand_callback();
  bus_expand9 : Subsystem  AncestorBlock=casper_library_flow_control/bus_expand  mask(bus_expand){mode=divisions of equal size, outputNum=2, outputWidth=18, outputBinaryPt=17, outputArithmeticType=1, show_format=off, outputToWorkspace=off, variablePrefix=out, outputToModelAsWell=on}
      mask prompts: outputNum "Number of outputs:"; outputWidth "Output width:"; outputBinaryPt "Output binary point position:"; outputArithmeticType "Output arithmetic type (ufix=0, fix=1, bool=2):"; show_format "Print format string?"; outputToWorkspace "Output to workspace?"; variablePrefix "Variable name prefix:"; outputToModelAsWell "Output to model as well?"
      mask help:
      | Expands a 'bus' made using a bus_create or Xilinx
      | concat block.
      | The input will be divided into the specified number
      | of outputs with the specified arithmetic types.
      | Divisions are made from most significant bit.
      mask init: same as s_c_nbe_m1k/bus_expand1
      settings: AttributesFormatString=2 outputs
      mask TypeOptions mode: divisions of equal size | divisions of arbitrary size
      mask Callback mode: bus_expand_callback();
      mask Callback outputWidth: bus_expand_callback();
      mask Callback outputToWorkspace: bus_expand_callback();
  edge_detect1 : Subsystem  AncestorBlock=casper_library_misc/edge_detect  mask(edge_detect){edge=Rising, polarity=Active High, x_in=[0 0.08 0.08 0.16 0.16 0.24 0.24 0.32 0.32 0.4], y_in=[-1 -1  1  1  1  1  1  1  1  1], x_out=[0.6 0.68 0.68 0.76 0.76 0.84 0.84 0.92 0.92 1], y_out=[-1 -1  1  1 -1 -1 -1 -1 -1 -1]}
      mask prompts: edge "Edge Type"; polarity "Output Polarity"; x_in "Input X Positions"; y_in "Input Y Positions"; x_out "Output X Positions"; y_out "Output Y Positions"
      mask help: Output is active for one-cycle after each edge of the specified type (i.e. rising, falling or both).
      mask init: same as s_c_nbe_m1k/edge_detect1
      settings: AttributesFormatString=|
      | rising edges
      | active high
      mask Help: Output is active for one-cycle after each edge of the specified type (i.e. rising, falling, or both).  Latency is zero.
      mask TypeOptions edge: Rising | Falling | Both
      mask TypeOptions polarity: Active High | Active Low
      mask Display:
      | plot(x_in_num,0.5+y_in_num*0.2);
      | plot(x_out_num,0.5+y_out_num*0.2);
  edge_detect10 : Subsystem  AncestorBlock=casper_library_misc/edge_detect  mask(edge_detect){edge=Rising, polarity=Active High, x_in=[0 0.08 0.08 0.16 0.16 0.24 0.24 0.32 0.32 0.4], y_in=[-1 -1  1  1  1  1  1  1  1  1], x_out=[0.6 0.68 0.68 0.76 0.76 0.84 0.84 0.92 0.92 1], y_out=[-1 -1  1  1 -1 -1 -1 -1 -1 -1]}
      mask prompts: edge "Edge Type"; polarity "Output Polarity"; x_in "Input X Positions"; y_in "Input Y Positions"; x_out "Output X Positions"; y_out "Output Y Positions"
      mask help: Output is active for one-cycle after each edge of the specified type (i.e. rising, falling or both).
      mask init: same as s_c_nbe_m1k/edge_detect1
      settings: AttributesFormatString=|
      | rising edges
      | active high
      mask Help: Output is active for one-cycle after each edge of the specified type (i.e. rising, falling, or both).  Latency is zero.
      mask TypeOptions edge: Rising | Falling | Both
      mask TypeOptions polarity: Active High | Active Low
      mask Display:
      | plot(x_in_num,0.5+y_in_num*0.2);
      | plot(x_out_num,0.5+y_out_num*0.2);
  edge_detect2 : Subsystem  AncestorBlock=casper_library_misc/edge_detect  mask(edge_detect){edge=Rising, polarity=Active High, x_in=[0 0.08 0.08 0.16 0.16 0.24 0.24 0.32 0.32 0.4], y_in=[-1 -1  1  1  1  1  1  1  1  1], x_out=[0.6 0.68 0.68 0.76 0.76 0.84 0.84 0.92 0.92 1], y_out=[-1 -1  1  1 -1 -1 -1 -1 -1 -1]}
      mask prompts: edge "Edge Type"; polarity "Output Polarity"; x_in "Input X Positions"; y_in "Input Y Positions"; x_out "Output X Positions"; y_out "Output Y Positions"
      mask help: Output is active for one-cycle after each edge of the specified type (i.e. rising, falling or both).
      mask init: same as s_c_nbe_m1k/edge_detect1
      settings: AttributesFormatString=|
      | rising edges
      | active high
      mask Help: Output is active for one-cycle after each edge of the specified type (i.e. rising, falling, or both).  Latency is zero.
      mask TypeOptions edge: Rising | Falling | Both
      mask TypeOptions polarity: Active High | Active Low
      mask Display:
      | plot(x_in_num,0.5+y_in_num*0.2);
      | plot(x_out_num,0.5+y_out_num*0.2);
  edge_detect3 : Subsystem  AncestorBlock=casper_library_misc/edge_detect  mask(edge_detect){edge=Falling, polarity=Active High, x_in=[0 0.08 0.08 0.16 0.16 0.24 0.24 0.32 0.32 0.4], y_in=[-1 -1  1  1  1  1  1  1  1  1], x_out=[0.6 0.68 0.68 0.76 0.76 0.84 0.84 0.92 0.92 1], y_out=[-1 -1  1  1 -1 -1 -1 -1 -1 -1]}
      mask prompts: edge "Edge Type"; polarity "Output Polarity"; x_in "Input X Positions"; y_in "Input Y Positions"; x_out "Output X Positions"; y_out "Output Y Positions"
      mask help: Output is active for one-cycle after each edge of the specified type (i.e. rising, falling or both).
      mask init: same as s_c_nbe_m1k/edge_detect1
      settings: AttributesFormatString=|
      | falling edges
      | active high
      mask Help: Output is active for one-cycle after each edge of the specified type (i.e. rising, falling, or both).  Latency is zero.
      mask TypeOptions edge: Rising | Falling | Both
      mask TypeOptions polarity: Active High | Active Low
      mask Display:
      | plot(x_in_num,0.5+y_in_num*0.2);
      | plot(x_out_num,0.5+y_out_num*0.2);
  edge_detect4 : Subsystem  AncestorBlock=casper_library_misc/edge_detect  mask(edge_detect){edge=Rising, polarity=Active High, x_in=[0 0.08 0.08 0.16 0.16 0.24 0.24 0.32 0.32 0.4], y_in=[-1 -1  1  1  1  1  1  1  1  1], x_out=[0.6 0.68 0.68 0.76 0.76 0.84 0.84 0.92 0.92 1], y_out=[-1 -1  1  1 -1 -1 -1 -1 -1 -1]}
      mask prompts: edge "Edge Type"; polarity "Output Polarity"; x_in "Input X Positions"; y_in "Input Y Positions"; x_out "Output X Positions"; y_out "Output Y Positions"
      mask help: Output is active for one-cycle after each edge of the specified type (i.e. rising, falling or both).
      mask init: same as s_c_nbe_m1k/edge_detect1
      settings: AttributesFormatString=|
      | rising edges
      | active high
      mask Help: Output is active for one-cycle after each edge of the specified type (i.e. rising, falling, or both).  Latency is zero.
      mask TypeOptions edge: Rising | Falling | Both
      mask TypeOptions polarity: Active High | Active Low
      mask Display:
      | plot(x_in_num,0.5+y_in_num*0.2);
      | plot(x_out_num,0.5+y_out_num*0.2);
  edge_detect5 : Subsystem  AncestorBlock=casper_library_misc/edge_detect  mask(edge_detect){edge=Rising, polarity=Active High, x_in=[0 0.08 0.08 0.16 0.16 0.24 0.24 0.32 0.32 0.4], y_in=[-1 -1  1  1  1  1  1  1  1  1], x_out=[0.6 0.68 0.68 0.76 0.76 0.84 0.84 0.92 0.92 1], y_out=[-1 -1  1  1 -1 -1 -1 -1 -1 -1]}
      mask prompts: edge "Edge Type"; polarity "Output Polarity"; x_in "Input X Positions"; y_in "Input Y Positions"; x_out "Output X Positions"; y_out "Output Y Positions"
      mask help: Output is active for one-cycle after each edge of the specified type (i.e. rising, falling or both).
      mask init: same as s_c_nbe_m1k/edge_detect1
      settings: AttributesFormatString=|
      | rising edges
      | active high
      mask Help: Output is active for one-cycle after each edge of the specified type (i.e. rising, falling, or both).  Latency is zero.
      mask TypeOptions edge: Rising | Falling | Both
      mask TypeOptions polarity: Active High | Active Low
      mask Display:
      | plot(x_in_num,0.5+y_in_num*0.2);
      | plot(x_out_num,0.5+y_out_num*0.2);
  edge_detect6 : Subsystem  AncestorBlock=casper_library_misc/edge_detect  mask(edge_detect){edge=Rising, polarity=Active High, x_in=[0 0.08 0.08 0.16 0.16 0.24 0.24 0.32 0.32 0.4], y_in=[-1 -1  1  1  1  1  1  1  1  1], x_out=[0.6 0.68 0.68 0.76 0.76 0.84 0.84 0.92 0.92 1], y_out=[-1 -1  1  1 -1 -1 -1 -1 -1 -1]}
      mask prompts: edge "Edge Type"; polarity "Output Polarity"; x_in "Input X Positions"; y_in "Input Y Positions"; x_out "Output X Positions"; y_out "Output Y Positions"
      mask help: Output is active for one-cycle after each edge of the specified type (i.e. rising, falling or both).
      mask init: same as s_c_nbe_m1k/edge_detect1
      settings: AttributesFormatString=|
      | rising edges
      | active high
      mask Help: Output is active for one-cycle after each edge of the specified type (i.e. rising, falling, or both).  Latency is zero.
      mask TypeOptions edge: Rising | Falling | Both
      mask TypeOptions polarity: Active High | Active Low
      mask Display:
      | plot(x_in_num,0.5+y_in_num*0.2);
      | plot(x_out_num,0.5+y_out_num*0.2);
  edge_detect7 : Subsystem  AncestorBlock=casper_library_misc/edge_detect  mask(edge_detect){edge=Rising, polarity=Active High, x_in=[0 0.08 0.08 0.16 0.16 0.24 0.24 0.32 0.32 0.4], y_in=[-1 -1  1  1  1  1  1  1  1  1], x_out=[0.6 0.68 0.68 0.76 0.76 0.84 0.84 0.92 0.92 1], y_out=[-1 -1  1  1 -1 -1 -1 -1 -1 -1]}
      mask prompts: edge "Edge Type"; polarity "Output Polarity"; x_in "Input X Positions"; y_in "Input Y Positions"; x_out "Output X Positions"; y_out "Output Y Positions"
      mask help: Output is active for one-cycle after each edge of the specified type (i.e. rising, falling or both).
      mask init: same as s_c_nbe_m1k/edge_detect1
      settings: AttributesFormatString=|
      | rising edges
      | active high
      mask Help: Output is active for one-cycle after each edge of the specified type (i.e. rising, falling, or both).  Latency is zero.
      mask TypeOptions edge: Rising | Falling | Both
      mask TypeOptions polarity: Active High | Active Low
      mask Display:
      | plot(x_in_num,0.5+y_in_num*0.2);
      | plot(x_out_num,0.5+y_out_num*0.2);
  edge_detect9 : Subsystem  AncestorBlock=casper_library_misc/edge_detect  mask(edge_detect){edge=Rising, polarity=Active High, x_in=[0 0.08 0.08 0.16 0.16 0.24 0.24 0.32 0.32 0.4], y_in=[-1 -1  1  1  1  1  1  1  1  1], x_out=[0.6 0.68 0.68 0.76 0.76 0.84 0.84 0.92 0.92 1], y_out=[-1 -1  1  1 -1 -1 -1 -1 -1 -1]}
      mask prompts: edge "Edge Type"; polarity "Output Polarity"; x_in "Input X Positions"; y_in "Input Y Positions"; x_out "Output X Positions"; y_out "Output Y Positions"
      mask help: Output is active for one-cycle after each edge of the specified type (i.e. rising, falling or both).
      mask init: same as s_c_nbe_m1k/edge_detect1
      settings: AttributesFormatString=|
      | rising edges
      | active high
      mask Help: Output is active for one-cycle after each edge of the specified type (i.e. rising, falling, or both).  Latency is zero.
      mask TypeOptions edge: Rising | Falling | Both
      mask TypeOptions polarity: Active High | Active Low
      mask Display:
      | plot(x_in_num,0.5+y_in_num*0.2);
      | plot(x_out_num,0.5+y_out_num*0.2);
  fft_ch_err : Subsystem  Tag=xps:sw_reg  AncestorBlock=xps_library/Memory/software_register  mask(swreg){io_dir=To Processor, io_delay=0, init_val=0, sample_period=1, names=reg, bitwidths=8, bin_pts=0, arith_types=0, sim_port=off, show_format=on}
      mask prompts: io_dir "I/O direction"; io_delay "I/O delay"; init_val "Initial Value"; sample_period "Sample period"; names "Bitfield names [msb...lsb]"; bitwidths "Bitfield widths"; bin_pts "Bitfield binary pts"; arith_types "Bitfield types, ufix=0, fix=1, bool=2"; sim_port "Provide sim input/output?"; show_format "Print format string?"
      mask help: A 32-bit software-accessible register. Can be divided into bitfields of varying widths and types using the fields in the block mask.
      mask init:
      | swreg_init(gcb)
      settings: AttributesFormatString=1output:uf8.0 = 8 bits
      mask TypeOptions io_dir: To Processor | From Processor
      mask Callback io_dir:
      | mask_enables = get_param(gcb, 'MaskEnables');
      | mask_names = get_param(gcb, 'MaskNames');
      | if strcmp(get_param(gcb, 'io_dir'), 'To Processor'),
      |     mask_enables{ismember(mask_names, 'sample_period')} = 'off';
      | else
      |     mask_enables{ismember(mask_names, 'sample_period')} = 'on';
      | end
      | set_param(gcb, 'MaskEnables', mask_enables);
      mask DialogControl ParameterTabVar0 Prompt: Setup
  fft_shift_change : Subsystem  Tag=xps:sw_reg  AncestorBlock=xps_library/Memory/software_register  mask(swreg){io_dir=To Processor, io_delay=0, init_val=0, sample_period=1, names=reg, bitwidths=32, bin_pts=0, arith_types=0, sim_port=off, show_format=on}
      mask prompts: io_dir "I/O direction"; io_delay "I/O delay"; init_val "Initial Value"; sample_period "Sample period"; names "Bitfield names [msb...lsb]"; bitwidths "Bitfield widths"; bin_pts "Bitfield binary pts"; arith_types "Bitfield types, ufix=0, fix=1, bool=2"; sim_port "Provide sim input/output?"; show_format "Print format string?"
      mask help: A 32-bit software-accessible register. Can be divided into bitfields of varying widths and types using the fields in the block mask.
      mask init:
      | swreg_init(gcb)
      settings: AttributesFormatString=1output:uf32.0 = 32 bits
      mask TypeOptions io_dir: To Processor | From Processor
      mask Callback io_dir:
      | mask_enables = get_param(gcb, 'MaskEnables');
      | mask_names = get_param(gcb, 'MaskNames');
      | if strcmp(get_param(gcb, 'io_dir'), 'To Processor'),
      |     mask_enables{ismember(mask_names, 'sample_period')} = 'off';
      | else
      |     mask_enables{ismember(mask_names, 'sample_period')} = 'on';
      | end
      | set_param(gcb, 'MaskEnables', mask_enables);
      mask DialogControl ParameterTabVar0 Prompt: Setup
  fft_shift_value : Subsystem  Tag=xps:sw_reg  AncestorBlock=xps_library/Memory/software_register  mask(swreg){io_dir=To Processor, io_delay=0, init_val=0, sample_period=1, names=reg, bitwidths=10, bin_pts=0, arith_types=0, sim_port=off, show_format=on}
      mask prompts: io_dir "I/O direction"; io_delay "I/O delay"; init_val "Initial Value"; sample_period "Sample period"; names "Bitfield names [msb...lsb]"; bitwidths "Bitfield widths"; bin_pts "Bitfield binary pts"; arith_types "Bitfield types, ufix=0, fix=1, bool=2"; sim_port "Provide sim input/output?"; show_format "Print format string?"
      mask help: A 32-bit software-accessible register. Can be divided into bitfields of varying widths and types using the fields in the block mask.
      mask init:
      | swreg_init(gcb)
      settings: AttributesFormatString=1output:uf10.0 = 10 bits
      mask TypeOptions io_dir: To Processor | From Processor
      mask Callback io_dir:
      | mask_enables = get_param(gcb, 'MaskEnables');
      | mask_names = get_param(gcb, 'MaskNames');
      | if strcmp(get_param(gcb, 'io_dir'), 'To Processor'),
      |     mask_enables{ismember(mask_names, 'sample_period')} = 'off';
      | else
      |     mask_enables{ismember(mask_names, 'sample_period')} = 'on';
      | end
      | set_param(gcb, 'MaskEnables', mask_enables);
      mask DialogControl ParameterTabVar0 Prompt: Setup
  fft_sync_cnt : Subsystem  Tag=xps:sw_reg  AncestorBlock=xps_library/Memory/software_register  mask(swreg){io_dir=To Processor, io_delay=0, init_val=0, sample_period=1, names=reg, bitwidths=11, bin_pts=0, arith_types=0, sim_port=off, show_format=on}
      mask prompts: io_dir "I/O direction"; io_delay "I/O delay"; init_val "Initial Value"; sample_period "Sample period"; names "Bitfield names [msb...lsb]"; bitwidths "Bitfield widths"; bin_pts "Bitfield binary pts"; arith_types "Bitfield types, ufix=0, fix=1, bool=2"; sim_port "Provide sim input/output?"; show_format "Print format string?"
      mask help: A 32-bit software-accessible register. Can be divided into bitfields of varying widths and types using the fields in the block mask.
      mask init:
      | swreg_init(gcb)
      settings: AttributesFormatString=1output:uf11.0 = 11 bits
      mask TypeOptions io_dir: To Processor | From Processor
      mask Callback io_dir:
      | mask_enables = get_param(gcb, 'MaskEnables');
      | mask_names = get_param(gcb, 'MaskNames');
      | if strcmp(get_param(gcb, 'io_dir'), 'To Processor'),
      |     mask_enables{ismember(mask_names, 'sample_period')} = 'off';
      | else
      |     mask_enables{ismember(mask_names, 'sample_period')} = 'on';
      | end
      | set_param(gcb, 'MaskEnables', mask_enables);
      mask DialogControl ParameterTabVar0 Prompt: Setup
  fir_sync_cnt : Subsystem  Tag=xps:sw_reg  AncestorBlock=xps_library/Memory/software_register  mask(swreg){io_dir=To Processor, io_delay=0, init_val=0, sample_period=1, names=reg, bitwidths=32, bin_pts=0, arith_types=0, sim_port=off, show_format=on}
      mask prompts: io_dir "I/O direction"; io_delay "I/O delay"; init_val "Initial Value"; sample_period "Sample period"; names "Bitfield names [msb...lsb]"; bitwidths "Bitfield widths"; bin_pts "Bitfield binary pts"; arith_types "Bitfield types, ufix=0, fix=1, bool=2"; sim_port "Provide sim input/output?"; show_format "Print format string?"
      mask help: A 32-bit software-accessible register. Can be divided into bitfields of varying widths and types using the fields in the block mask.
      mask init:
      | swreg_init(gcb)
      settings: AttributesFormatString=1output:uf32.0 = 32 bits
      mask TypeOptions io_dir: To Processor | From Processor
      mask Callback io_dir:
      | mask_enables = get_param(gcb, 'MaskEnables');
      | mask_names = get_param(gcb, 'MaskNames');
      | if strcmp(get_param(gcb, 'io_dir'), 'To Processor'),
      |     mask_enables{ismember(mask_names, 'sample_period')} = 'off';
      | else
      |     mask_enables{ismember(mask_names, 'sample_period')} = 'on';
      | end
      | set_param(gcb, 'MaskEnables', mask_enables);
      mask DialogControl ParameterTabVar0 Prompt: Setup
  lsb_0 : xbsIndex_r4/Slice  nbits=1  boolean_output=on  mode=Lower Bit Location + Width  bit1=0  base1=MSB of Input  bit0=0  base0=LSB of Input  dbl_ovrd=off  block_type=slice
  lsb_1 : xbsIndex_r4/Slice  nbits=1  boolean_output=on  mode=Lower Bit Location + Width  bit1=0  base1=MSB of Input  bit0=1  base0=LSB of Input  dbl_ovrd=off  block_type=slice
  pfb_fir_generic : Subsystem  Tag=casper:pfb_fir_generic  AncestorBlock=casper_library_pfbs/pfb_fir_generic  mask(pfb_fir_generic){n_streams=1, PFBSize=fft_stages-1, TotalTaps=n_taps, n_inputs=0, BitWidthIn=18, BitWidthOut=18, CoeffBitWidth=18, complex=on, async=on, floating_point=off, float_type=single, frac_width=0, exp_width=0, WindowType=hann, quantization=Round  (unbiased: +/- Inf), fwidth=1, coeffs_bram_optimization=Speed, delays_bram_optimization=Speed, add_latency=7, mult_latency=7, bram_latency=7, fan_latency=4, conv_latency=4, fixed_float_latency=0}
      mask prompts: n_streams "Number input streams?"; PFBSize "Size of PFB: (2^? pnts)"; TotalTaps "Total Number of Taps:"; n_inputs "Number of Simultaneous Inputs: (2^?)"; BitWidthIn "Input Bitwidth:"; BitWidthOut "Output Bitwidth:"; CoeffBitWidth "Coefficient Bitwidth:"; complex "Complex data inputs"; async "Asynchronous operation"; floating_point "floating point"; float_type "float type"; frac_width "fraction width"; exp_width "exponent width"; WindowType "Windowing Function:"; quantization "Quantization Behavior"; fwidth "Bin Width Scaling (normal=1)"; coeffs_bram_optimization "Coefficient BRAMs optimization"; delays_bram_optimization "Delay BRAMs optimization"; add_latency "Add Latency"; mult_latency "Mult Latency"; bram_latency "BRAM Latency"; fan_latency "Fanout Latency"; conv_latency "Convert latency"; fixed_float_latency "Fixed to float latency"
      mask init:
      | % pfb_fir_generic_init(gcb, ...
      | %     'n_streams', n_streams, ...
      | %     'PFBSize', PFBSize, ...
      | %     'TotalTaps', TotalTaps, ...
      | %     'WindowType', WindowType, ...
      | %     'n_inputs', n_inputs, ...
      | %     'complex', complex, ...
      | %     'BitWidthIn', BitWidthIn, ...
      | %     'BitWidthOut', BitWidthOut, ...
      | %     'CoeffBitWidth', CoeffBitWidth, ...
      | %     'floating_point', floating_point, ...
      | %     'float_type', float_type, ...
      | %     'exp_width', exp_width, ...
      | %     'frac_width', frac_width, ... 
      | %     'fixed_float_latency', fixed_float_latency, ...
      | %     'async', async, ...
      | %     'add_latency', add_latency, ...
      | %     'mult_latency', mult_latency, ...
      | %     'bram_latency', bram_latency, ...
      | %     'fan_latency', fan_latency, ...
      | %     'conv_latency', conv_latency, ...
      | %     'quantization', quantization, ...
      | %     'fwidth', fwidth, ...
      | %     'coeffs_bram_optimization', coeffs_bram_optimization, ...
      | %     'delays_bram_optimization', delays_bram_optimization);
      mask Callback TotalTaps:
      | %num_taps = eval(get_param(gcb, 'TotalTaps'));
      | %old_vec = eval(get_param(gcb, 'mult_spec'));
      | 
      | %vec = 2.*ones(1,num_taps);
      | %old_size = length(old_vec);
      | 
      | %if(old_size <= num_taps),
      | %   new_size = old_size;
      | %else,
      | %    new_size = num_taps;
      | %end
      | 
      | %for n = 1:new_size, vec(n) = old_vec(n); end
      | %set_param(gcb, 'mult_spec', mat2str(vec));
      mask Callback floating_point:
      | onoff = get_param(gcb, 'floating_point');
      | if strcmp(onoff,'on')
      |     enable_fixpt = 'off'
      |     set_param_state(gcb, 'float_type', 'on')
      |     set_param_state(gcb, 'fixed_float_latency', 'on')
      | 
      | 
      |     f_type = get_param(gcb, 'float_type')
      |     if strcmp(f_type,'custom')
      |         set_param_state(gcb, 'exp_width', 'on')
      |         set_param_state(gcb, 'frac_width', 'on')
      |     else
      |         set_param_state(gcb, 'exp_width', 'off')
      |         set_param_state(gcb, 'frac_width', 'off')
      |     end
      | 
      | else
      |     enable_fixpt = 'on'
      |     set_param_state(gcb, 'float_type', 'off')
      |     set_param_state(gcb, 'exp_width', 'off')
      |     set_param_state(gcb, 'frac_width', 'off')
      |     set_param_state(gcb, 'fixed_float_latency', 'off')
      | end
      | 
      | set_param_state(gcb, 'BitWidthIn', enable_fixpt)
      | set_param_state(gcb, 'BitWidthOut', enable_fixpt)
      | %set_param_state(gcb, 'CoeffBitWidth', enable_fixpt)
      mask TypeOptions float_type: single | custom
      mask Callback float_type:
      | f_type = get_param(gcb, 'float_type')
      | if strcmp(f_type,'custom')
      |     set_param_state(gcb, 'exp_width', 'on')
      |     set_param_state(gcb, 'frac_width', 'on')
      | else
      |     set_param_state(gcb, 'exp_width', 'off')
      |     set_param_state(gcb, 'frac_width', 'off')
      | end
      mask TypeOptions WindowType: bartlett | barthannwin | blackman | blackmanharris | bohamwin | chebwin | flattopwin | gausswin | hamming | hann | kaiser | nuttallwin | parzenwin | rectwin | tukeywin | triang | userwindow
      mask TypeOptions quantization: Truncate | Round  (unbiased: +/- Inf) | Round  (unbiased: Even Values)
      mask Callback fwidth:
      | %num_taps = eval(get_param(gcb, 'TotalTaps'));
      | %old_vec = eval(get_param(gcb, 'mult_spec'));
      | 
      | %vec = 2.*ones(1,num_taps);
      | %old_size = length(old_vec);
      | 
      | %if(old_size <= num_taps),
      | %    new_size = old_size;
      | %else,
      | %    new_size = num_taps;
      | %end
      | 
      | %for n = 1:new_size, vec(n) = old_vec(n); end
      | %set_param(gcb, 'mult_spec', mat2str(vec));
      mask TypeOptions coeffs_bram_optimization: Area | Speed
      mask TypeOptions delays_bram_optimization: Area | Speed
  pfb_fir_generic1 : Subsystem  Tag=casper:pfb_fir_generic  AncestorBlock=casper_library_pfbs/pfb_fir_generic  mask(pfb_fir_generic){n_streams=1, PFBSize=fft_stages-1, TotalTaps=n_taps, n_inputs=0, BitWidthIn=18, BitWidthOut=18, CoeffBitWidth=18, complex=on, async=on, floating_point=off, float_type=single, frac_width=0, exp_width=0, WindowType=hann, quantization=Round  (unbiased: +/- Inf), fwidth=1, coeffs_bram_optimization=Speed, delays_bram_optimization=Speed, add_latency=7, mult_latency=7, bram_latency=7, fan_latency=4, conv_latency=4, fixed_float_latency=0}
      mask prompts: n_streams "Number input streams?"; PFBSize "Size of PFB: (2^? pnts)"; TotalTaps "Total Number of Taps:"; n_inputs "Number of Simultaneous Inputs: (2^?)"; BitWidthIn "Input Bitwidth:"; BitWidthOut "Output Bitwidth:"; CoeffBitWidth "Coefficient Bitwidth:"; complex "Complex data inputs"; async "Asynchronous operation"; floating_point "floating point"; float_type "float type"; frac_width "fraction width"; exp_width "exponent width"; WindowType "Windowing Function:"; quantization "Quantization Behavior"; fwidth "Bin Width Scaling (normal=1)"; coeffs_bram_optimization "Coefficient BRAMs optimization"; delays_bram_optimization "Delay BRAMs optimization"; add_latency "Add Latency"; mult_latency "Mult Latency"; bram_latency "BRAM Latency"; fan_latency "Fanout Latency"; conv_latency "Convert latency"; fixed_float_latency "Fixed to float latency"
      mask init: same as s_c_nbe_m1k/nb_pfb/pfb_fir_generic
      mask Callback TotalTaps:
      | %num_taps = eval(get_param(gcb, 'TotalTaps'));
      | %old_vec = eval(get_param(gcb, 'mult_spec'));
      | 
      | %vec = 2.*ones(1,num_taps);
      | %old_size = length(old_vec);
      | 
      | %if(old_size <= num_taps),
      | %   new_size = old_size;
      | %else,
      | %    new_size = num_taps;
      | %end
      | 
      | %for n = 1:new_size, vec(n) = old_vec(n); end
      | %set_param(gcb, 'mult_spec', mat2str(vec));
      mask Callback floating_point:
      | onoff = get_param(gcb, 'floating_point');
      | if strcmp(onoff,'on')
      |     enable_fixpt = 'off'
      |     set_param_state(gcb, 'float_type', 'on')
      |     set_param_state(gcb, 'fixed_float_latency', 'on')
      | 
      | 
      |     f_type = get_param(gcb, 'float_type')
      |     if strcmp(f_type,'custom')
      |         set_param_state(gcb, 'exp_width', 'on')
      |         set_param_state(gcb, 'frac_width', 'on')
      |     else
      |         set_param_state(gcb, 'exp_width', 'off')
      |         set_param_state(gcb, 'frac_width', 'off')
      |     end
      | 
      | else
      |     enable_fixpt = 'on'
      |     set_param_state(gcb, 'float_type', 'off')
      |     set_param_state(gcb, 'exp_width', 'off')
      |     set_param_state(gcb, 'frac_width', 'off')
      |     set_param_state(gcb, 'fixed_float_latency', 'off')
      | end
      | 
      | set_param_state(gcb, 'BitWidthIn', enable_fixpt)
      | set_param_state(gcb, 'BitWidthOut', enable_fixpt)
      | %set_param_state(gcb, 'CoeffBitWidth', enable_fixpt)
      mask TypeOptions float_type: single | custom
      mask Callback float_type:
      | f_type = get_param(gcb, 'float_type')
      | if strcmp(f_type,'custom')
      |     set_param_state(gcb, 'exp_width', 'on')
      |     set_param_state(gcb, 'frac_width', 'on')
      | else
      |     set_param_state(gcb, 'exp_width', 'off')
      |     set_param_state(gcb, 'frac_width', 'off')
      | end
      mask TypeOptions WindowType: bartlett | barthannwin | blackman | blackmanharris | bohamwin | chebwin | flattopwin | gausswin | hamming | hann | kaiser | nuttallwin | parzenwin | rectwin | tukeywin | triang | userwindow
      mask TypeOptions quantization: Truncate | Round  (unbiased: +/- Inf) | Round  (unbiased: Even Values)
      mask Callback fwidth:
      | %num_taps = eval(get_param(gcb, 'TotalTaps'));
      | %old_vec = eval(get_param(gcb, 'mult_spec'));
      | 
      | %vec = 2.*ones(1,num_taps);
      | %old_size = length(old_vec);
      | 
      | %if(old_size <= num_taps),
      | %    new_size = old_size;
      | %else,
      | %    new_size = num_taps;
      | %end
      | 
      | %for n = 1:new_size, vec(n) = old_vec(n); end
      | %set_param(gcb, 'mult_spec', mat2str(vec));
      mask TypeOptions coeffs_bram_optimization: Area | Speed
      mask TypeOptions delays_bram_optimization: Area | Speed
  pipeline1 : Subsystem  AncestorBlock=casper_library_delays/pipeline  mask(pipeline){latency=2}
      mask help:
      | An explicitly laid-out delay line to avoid mapping to SRL16s
      | for use in pipelining to help achieve timing closure.
      mask init:
      | pipeline_init(gcb,'latency',latency);
      settings: AttributesFormatString=Latency = %<latency>
      mask Display:
      | port_label('input', 1, 'd');
      | port_label('output', 1, 'q');
      | disp(['Z^-', num2str(latency)]);
  pipeline10 : Subsystem  AncestorBlock=casper_library_delays/pipeline  mask(pipeline){latency=4}
      mask help:
      | An explicitly laid-out delay line to avoid mapping to SRL16s
      | for use in pipelining to help achieve timing closure.
      mask init:
      | pipeline_init(gcb,'latency',latency);
      settings: AttributesFormatString=Latency = %<latency>
      mask Display:
      | port_label('input', 1, 'd');
      | port_label('output', 1, 'q');
      | disp(['Z^-', num2str(latency)]);
  pipeline11 : Subsystem  AncestorBlock=casper_library_delays/pipeline  mask(pipeline){latency=5}
      mask help:
      | An explicitly laid-out delay line to avoid mapping to SRL16s
      | for use in pipelining to help achieve timing closure.
      mask init:
      | pipeline_init(gcb,'latency',latency);
      settings: AttributesFormatString=Latency = %<latency>
      mask Display:
      | port_label('input', 1, 'd');
      | port_label('output', 1, 'q');
      | disp(['Z^-', num2str(latency)]);
  pipeline110 : Subsystem  AncestorBlock=casper_library_delays/pipeline  mask(pipeline){latency=2}
      mask help:
      | An explicitly laid-out delay line to avoid mapping to SRL16s
      | for use in pipelining to help achieve timing closure.
      mask init:
      | pipeline_init(gcb,'latency',latency);
      settings: AttributesFormatString=Latency = %<latency>
      mask Display:
      | port_label('input', 1, 'd');
      | port_label('output', 1, 'q');
      | disp(['Z^-', num2str(latency)]);
  pipeline117 : Subsystem  AncestorBlock=casper_library_delays/pipeline  mask(pipeline){latency=2}
      mask help:
      | An explicitly laid-out delay line to avoid mapping to SRL16s
      | for use in pipelining to help achieve timing closure.
      mask init:
      | pipeline_init(gcb,'latency',latency);
      settings: AttributesFormatString=Latency = %<latency>
      mask Display:
      | port_label('input', 1, 'd');
      | port_label('output', 1, 'q');
      | disp(['Z^-', num2str(latency)]);
  pipeline12 : Subsystem  AncestorBlock=casper_library_delays/pipeline  mask(pipeline){latency=2}
      mask help:
      | An explicitly laid-out delay line to avoid mapping to SRL16s
      | for use in pipelining to help achieve timing closure.
      mask init:
      | pipeline_init(gcb,'latency',latency);
      settings: AttributesFormatString=Latency = %<latency>
      mask Display:
      | port_label('input', 1, 'd');
      | port_label('output', 1, 'q');
      | disp(['Z^-', num2str(latency)]);
  pipeline122 : Subsystem  AncestorBlock=casper_library_delays/pipeline  mask(pipeline){latency=2}
      mask help:
      | An explicitly laid-out delay line to avoid mapping to SRL16s
      | for use in pipelining to help achieve timing closure.
      mask init:
      | pipeline_init(gcb,'latency',latency);
      settings: AttributesFormatString=Latency = %<latency>
      mask Display:
      | port_label('input', 1, 'd');
      | port_label('output', 1, 'q');
      | disp(['Z^-', num2str(latency)]);
  pipeline123 : Subsystem  AncestorBlock=casper_library_delays/pipeline  mask(pipeline){latency=2}
      mask help:
      | An explicitly laid-out delay line to avoid mapping to SRL16s
      | for use in pipelining to help achieve timing closure.
      mask init:
      | pipeline_init(gcb,'latency',latency);
      settings: AttributesFormatString=Latency = %<latency>
      mask Display:
      | port_label('input', 1, 'd');
      | port_label('output', 1, 'q');
      | disp(['Z^-', num2str(latency)]);
  pipeline124 : Subsystem  AncestorBlock=casper_library_delays/pipeline  mask(pipeline){latency=2}
      mask help:
      | An explicitly laid-out delay line to avoid mapping to SRL16s
      | for use in pipelining to help achieve timing closure.
      mask init:
      | pipeline_init(gcb,'latency',latency);
      settings: AttributesFormatString=Latency = %<latency>
      mask Display:
      | port_label('input', 1, 'd');
      | port_label('output', 1, 'q');
      | disp(['Z^-', num2str(latency)]);
  pipeline126 : Subsystem  AncestorBlock=casper_library_delays/pipeline  mask(pipeline){latency=2}
      mask help:
      | An explicitly laid-out delay line to avoid mapping to SRL16s
      | for use in pipelining to help achieve timing closure.
      mask init:
      | pipeline_init(gcb,'latency',latency);
      settings: AttributesFormatString=Latency = %<latency>
      mask Display:
      | port_label('input', 1, 'd');
      | port_label('output', 1, 'q');
      | disp(['Z^-', num2str(latency)]);
  pipeline127 : Subsystem  AncestorBlock=casper_library_delays/pipeline  mask(pipeline){latency=2}
      mask help:
      | An explicitly laid-out delay line to avoid mapping to SRL16s
      | for use in pipelining to help achieve timing closure.
      mask init:
      | pipeline_init(gcb,'latency',latency);
      settings: AttributesFormatString=Latency = %<latency>
      mask Display:
      | port_label('input', 1, 'd');
      | port_label('output', 1, 'q');
      | disp(['Z^-', num2str(latency)]);
  pipeline128 : Subsystem  AncestorBlock=casper_library_delays/pipeline  mask(pipeline){latency=2}
      mask help:
      | An explicitly laid-out delay line to avoid mapping to SRL16s
      | for use in pipelining to help achieve timing closure.
      mask init:
      | pipeline_init(gcb,'latency',latency);
      settings: AttributesFormatString=Latency = %<latency>
      mask Display:
      | port_label('input', 1, 'd');
      | port_label('output', 1, 'q');
      | disp(['Z^-', num2str(latency)]);
  pipeline129 : Subsystem  AncestorBlock=casper_library_delays/pipeline  mask(pipeline){latency=2}
      mask help:
      | An explicitly laid-out delay line to avoid mapping to SRL16s
      | for use in pipelining to help achieve timing closure.
      mask init:
      | pipeline_init(gcb,'latency',latency);
      settings: AttributesFormatString=Latency = %<latency>
      mask Display:
      | port_label('input', 1, 'd');
      | port_label('output', 1, 'q');
      | disp(['Z^-', num2str(latency)]);
  pipeline13 : Subsystem  AncestorBlock=casper_library_delays/pipeline  mask(pipeline){latency=1}
      mask help:
      | An explicitly laid-out delay line to avoid mapping to SRL16s
      | for use in pipelining to help achieve timing closure.
      mask init:
      | pipeline_init(gcb,'latency',latency);
      settings: AttributesFormatString=Latency = %<latency>
      mask Display:
      | port_label('input', 1, 'd');
      | port_label('output', 1, 'q');
      | disp(['Z^-', num2str(latency)]);
  pipeline131 : Subsystem  AncestorBlock=casper_library_delays/pipeline  mask(pipeline){latency=2}
      mask help:
      | An explicitly laid-out delay line to avoid mapping to SRL16s
      | for use in pipelining to help achieve timing closure.
      mask init:
      | pipeline_init(gcb,'latency',latency);
      settings: AttributesFormatString=Latency = %<latency>
      mask Display:
      | port_label('input', 1, 'd');
      | port_label('output', 1, 'q');
      | disp(['Z^-', num2str(latency)]);
  pipeline132 : Subsystem  AncestorBlock=casper_library_delays/pipeline  mask(pipeline){latency=2}
      mask help:
      | An explicitly laid-out delay line to avoid mapping to SRL16s
      | for use in pipelining to help achieve timing closure.
      mask init:
      | pipeline_init(gcb,'latency',latency);
      settings: AttributesFormatString=Latency = %<latency>
      mask Display:
      | port_label('input', 1, 'd');
      | port_label('output', 1, 'q');
      | disp(['Z^-', num2str(latency)]);
  pipeline14 : Subsystem  AncestorBlock=casper_library_delays/pipeline  mask(pipeline){latency=2}
      mask help:
      | An explicitly laid-out delay line to avoid mapping to SRL16s
      | for use in pipelining to help achieve timing closure.
      mask init:
      | pipeline_init(gcb,'latency',latency);
      settings: AttributesFormatString=Latency = %<latency>
      mask Display:
      | port_label('input', 1, 'd');
      | port_label('output', 1, 'q');
      | disp(['Z^-', num2str(latency)]);
  pipeline15 : Subsystem  AncestorBlock=casper_library_delays/pipeline  mask(pipeline){latency=2}
      mask help:
      | An explicitly laid-out delay line to avoid mapping to SRL16s
      | for use in pipelining to help achieve timing closure.
      mask init:
      | pipeline_init(gcb,'latency',latency);
      settings: AttributesFormatString=Latency = %<latency>
      mask Display:
      | port_label('input', 1, 'd');
      | port_label('output', 1, 'q');
      | disp(['Z^-', num2str(latency)]);
  pipeline16 : Subsystem  AncestorBlock=casper_library_delays/pipeline  mask(pipeline){latency=2}
      mask help:
      | An explicitly laid-out delay line to avoid mapping to SRL16s
      | for use in pipelining to help achieve timing closure.
      mask init:
      | pipeline_init(gcb,'latency',latency);
      settings: AttributesFormatString=Latency = %<latency>
      mask Display:
      | port_label('input', 1, 'd');
      | port_label('output', 1, 'q');
      | disp(['Z^-', num2str(latency)]);
  pipeline17 : Subsystem  AncestorBlock=casper_library_delays/pipeline  mask(pipeline){latency=2}
      mask help:
      | An explicitly laid-out delay line to avoid mapping to SRL16s
      | for use in pipelining to help achieve timing closure.
      mask init:
      | pipeline_init(gcb,'latency',latency);
      settings: AttributesFormatString=Latency = %<latency>
      mask Display:
      | port_label('input', 1, 'd');
      | port_label('output', 1, 'q');
      | disp(['Z^-', num2str(latency)]);
  pipeline18 : Subsystem  AncestorBlock=casper_library_delays/pipeline  mask(pipeline){latency=2}
      mask help:
      | An explicitly laid-out delay line to avoid mapping to SRL16s
      | for use in pipelining to help achieve timing closure.
      mask init:
      | pipeline_init(gcb,'latency',latency);
      settings: AttributesFormatString=Latency = %<latency>
      mask Display:
      | port_label('input', 1, 'd');
      | port_label('output', 1, 'q');
      | disp(['Z^-', num2str(latency)]);
  pipeline19 : Subsystem  AncestorBlock=casper_library_delays/pipeline  mask(pipeline){latency=2}
      mask help:
      | An explicitly laid-out delay line to avoid mapping to SRL16s
      | for use in pipelining to help achieve timing closure.
      mask init:
      | pipeline_init(gcb,'latency',latency);
      settings: AttributesFormatString=Latency = %<latency>
      mask Display:
      | port_label('input', 1, 'd');
      | port_label('output', 1, 'q');
      | disp(['Z^-', num2str(latency)]);
  pipeline2 : Subsystem  AncestorBlock=casper_library_delays/pipeline  mask(pipeline){latency=2}
      mask help:
      | An explicitly laid-out delay line to avoid mapping to SRL16s
      | for use in pipelining to help achieve timing closure.
      mask init:
      | pipeline_init(gcb,'latency',latency);
      settings: AttributesFormatString=Latency = %<latency>
      mask Display:
      | port_label('input', 1, 'd');
      | port_label('output', 1, 'q');
      | disp(['Z^-', num2str(latency)]);
  pipeline20 : Subsystem  AncestorBlock=casper_library_delays/pipeline  mask(pipeline){latency=2}
      mask help:
      | An explicitly laid-out delay line to avoid mapping to SRL16s
      | for use in pipelining to help achieve timing closure.
      mask init:
      | pipeline_init(gcb,'latency',latency);
      settings: AttributesFormatString=Latency = %<latency>
      mask Display:
      | port_label('input', 1, 'd');
      | port_label('output', 1, 'q');
      | disp(['Z^-', num2str(latency)]);
  pipeline21 : Subsystem  AncestorBlock=casper_library_delays/pipeline  mask(pipeline){latency=2}
      mask help:
      | An explicitly laid-out delay line to avoid mapping to SRL16s
      | for use in pipelining to help achieve timing closure.
      mask init:
      | pipeline_init(gcb,'latency',latency);
      settings: AttributesFormatString=Latency = %<latency>
      mask Display:
      | port_label('input', 1, 'd');
      | port_label('output', 1, 'q');
      | disp(['Z^-', num2str(latency)]);
  pipeline22 : Subsystem  AncestorBlock=casper_library_delays/pipeline  mask(pipeline){latency=2}
      mask help:
      | An explicitly laid-out delay line to avoid mapping to SRL16s
      | for use in pipelining to help achieve timing closure.
      mask init:
      | pipeline_init(gcb,'latency',latency);
      settings: AttributesFormatString=Latency = %<latency>
      mask Display:
      | port_label('input', 1, 'd');
      | port_label('output', 1, 'q');
      | disp(['Z^-', num2str(latency)]);
  pipeline229 : Subsystem  AncestorBlock=casper_library_delays/pipeline  mask(pipeline){latency=2}
      mask help:
      | An explicitly laid-out delay line to avoid mapping to SRL16s
      | for use in pipelining to help achieve timing closure.
      mask init:
      | pipeline_init(gcb,'latency',latency);
      settings: AttributesFormatString=Latency = %<latency>
      mask Display:
      | port_label('input', 1, 'd');
      | port_label('output', 1, 'q');
      | disp(['Z^-', num2str(latency)]);
  pipeline23 : Subsystem  AncestorBlock=casper_library_delays/pipeline  mask(pipeline){latency=2}
      mask help:
      | An explicitly laid-out delay line to avoid mapping to SRL16s
      | for use in pipelining to help achieve timing closure.
      mask init:
      | pipeline_init(gcb,'latency',latency);
      settings: AttributesFormatString=Latency = %<latency>
      mask Display:
      | port_label('input', 1, 'd');
      | port_label('output', 1, 'q');
      | disp(['Z^-', num2str(latency)]);
  pipeline230 : Subsystem  AncestorBlock=casper_library_delays/pipeline  mask(pipeline){latency=2}
      mask help:
      | An explicitly laid-out delay line to avoid mapping to SRL16s
      | for use in pipelining to help achieve timing closure.
      mask init:
      | pipeline_init(gcb,'latency',latency);
      settings: AttributesFormatString=Latency = %<latency>
      mask Display:
      | port_label('input', 1, 'd');
      | port_label('output', 1, 'q');
      | disp(['Z^-', num2str(latency)]);
  pipeline24 : Subsystem  AncestorBlock=casper_library_delays/pipeline  mask(pipeline){latency=2}
      mask help:
      | An explicitly laid-out delay line to avoid mapping to SRL16s
      | for use in pipelining to help achieve timing closure.
      mask init:
      | pipeline_init(gcb,'latency',latency);
      settings: AttributesFormatString=Latency = %<latency>
      mask Display:
      | port_label('input', 1, 'd');
      | port_label('output', 1, 'q');
      | disp(['Z^-', num2str(latency)]);
  pipeline25 : Subsystem  AncestorBlock=casper_library_delays/pipeline  mask(pipeline){latency=5}
      mask help:
      | An explicitly laid-out delay line to avoid mapping to SRL16s
      | for use in pipelining to help achieve timing closure.
      mask init:
      | pipeline_init(gcb,'latency',latency);
      settings: AttributesFormatString=Latency = %<latency>
      mask Display:
      | port_label('input', 1, 'd');
      | port_label('output', 1, 'q');
      | disp(['Z^-', num2str(latency)]);
  pipeline26 : Subsystem  AncestorBlock=casper_library_delays/pipeline  mask(pipeline){latency=1}
      mask help:
      | An explicitly laid-out delay line to avoid mapping to SRL16s
      | for use in pipelining to help achieve timing closure.
      mask init:
      | pipeline_init(gcb,'latency',latency);
      settings: AttributesFormatString=Latency = %<latency>
      mask Display:
      | port_label('input', 1, 'd');
      | port_label('output', 1, 'q');
      | disp(['Z^-', num2str(latency)]);
  pipeline27 : Subsystem  AncestorBlock=casper_library_delays/pipeline  mask(pipeline){latency=2}
      mask help:
      | An explicitly laid-out delay line to avoid mapping to SRL16s
      | for use in pipelining to help achieve timing closure.
      mask init:
      | pipeline_init(gcb,'latency',latency);
      settings: AttributesFormatString=Latency = %<latency>
      mask Display:
      | port_label('input', 1, 'd');
      | port_label('output', 1, 'q');
      | disp(['Z^-', num2str(latency)]);
  pipeline28 : Subsystem  AncestorBlock=casper_library_delays/pipeline  mask(pipeline){latency=2}
      mask help:
      | An explicitly laid-out delay line to avoid mapping to SRL16s
      | for use in pipelining to help achieve timing closure.
      mask init:
      | pipeline_init(gcb,'latency',latency);
      settings: AttributesFormatString=Latency = %<latency>
      mask Display:
      | port_label('input', 1, 'd');
      | port_label('output', 1, 'q');
      | disp(['Z^-', num2str(latency)]);
  pipeline29 : Subsystem  AncestorBlock=casper_library_delays/pipeline  mask(pipeline){latency=2}
      mask help:
      | An explicitly laid-out delay line to avoid mapping to SRL16s
      | for use in pipelining to help achieve timing closure.
      mask init:
      | pipeline_init(gcb,'latency',latency);
      settings: AttributesFormatString=Latency = %<latency>
      mask Display:
      | port_label('input', 1, 'd');
      | port_label('output', 1, 'q');
      | disp(['Z^-', num2str(latency)]);
  pipeline3 : Subsystem  AncestorBlock=casper_library_delays/pipeline  mask(pipeline){latency=2}
      mask help:
      | An explicitly laid-out delay line to avoid mapping to SRL16s
      | for use in pipelining to help achieve timing closure.
      mask init:
      | pipeline_init(gcb,'latency',latency);
      settings: AttributesFormatString=Latency = %<latency>
      mask Display:
      | port_label('input', 1, 'd');
      | port_label('output', 1, 'q');
      | disp(['Z^-', num2str(latency)]);
  pipeline30 : Subsystem  AncestorBlock=casper_library_delays/pipeline  mask(pipeline){latency=2}
      mask help:
      | An explicitly laid-out delay line to avoid mapping to SRL16s
      | for use in pipelining to help achieve timing closure.
      mask init:
      | pipeline_init(gcb,'latency',latency);
      settings: AttributesFormatString=Latency = %<latency>
      mask Display:
      | port_label('input', 1, 'd');
      | port_label('output', 1, 'q');
      | disp(['Z^-', num2str(latency)]);
  pipeline31 : Subsystem  AncestorBlock=casper_library_delays/pipeline  mask(pipeline){latency=2}
      mask help:
      | An explicitly laid-out delay line to avoid mapping to SRL16s
      | for use in pipelining to help achieve timing closure.
      mask init:
      | pipeline_init(gcb,'latency',latency);
      settings: AttributesFormatString=Latency = %<latency>
      mask Display:
      | port_label('input', 1, 'd');
      | port_label('output', 1, 'q');
      | disp(['Z^-', num2str(latency)]);
  pipeline32 : Subsystem  AncestorBlock=casper_library_delays/pipeline  mask(pipeline){latency=2}
      mask help:
      | An explicitly laid-out delay line to avoid mapping to SRL16s
      | for use in pipelining to help achieve timing closure.
      mask init:
      | pipeline_init(gcb,'latency',latency);
      settings: AttributesFormatString=Latency = %<latency>
      mask Display:
      | port_label('input', 1, 'd');
      | port_label('output', 1, 'q');
      | disp(['Z^-', num2str(latency)]);
  pipeline33 : Subsystem  AncestorBlock=casper_library_delays/pipeline  mask(pipeline){latency=2}
      mask help:
      | An explicitly laid-out delay line to avoid mapping to SRL16s
      | for use in pipelining to help achieve timing closure.
      mask init:
      | pipeline_init(gcb,'latency',latency);
      settings: AttributesFormatString=Latency = %<latency>
      mask Display:
      | port_label('input', 1, 'd');
      | port_label('output', 1, 'q');
      | disp(['Z^-', num2str(latency)]);
  pipeline34 : Subsystem  AncestorBlock=casper_library_delays/pipeline  mask(pipeline){latency=2}
      mask help:
      | An explicitly laid-out delay line to avoid mapping to SRL16s
      | for use in pipelining to help achieve timing closure.
      mask init:
      | pipeline_init(gcb,'latency',latency);
      settings: AttributesFormatString=Latency = %<latency>
      mask Display:
      | port_label('input', 1, 'd');
      | port_label('output', 1, 'q');
      | disp(['Z^-', num2str(latency)]);
  pipeline35 : Subsystem  AncestorBlock=casper_library_delays/pipeline  mask(pipeline){latency=2}
      mask help:
      | An explicitly laid-out delay line to avoid mapping to SRL16s
      | for use in pipelining to help achieve timing closure.
      mask init:
      | pipeline_init(gcb,'latency',latency);
      settings: AttributesFormatString=Latency = %<latency>
      mask Display:
      | port_label('input', 1, 'd');
      | port_label('output', 1, 'q');
      | disp(['Z^-', num2str(latency)]);
  pipeline36 : Subsystem  AncestorBlock=casper_library_delays/pipeline  mask(pipeline){latency=2}
      mask help:
      | An explicitly laid-out delay line to avoid mapping to SRL16s
      | for use in pipelining to help achieve timing closure.
      mask init:
      | pipeline_init(gcb,'latency',latency);
      settings: AttributesFormatString=Latency = %<latency>
      mask Display:
      | port_label('input', 1, 'd');
      | port_label('output', 1, 'q');
      | disp(['Z^-', num2str(latency)]);
  pipeline37 : Subsystem  AncestorBlock=casper_library_delays/pipeline  mask(pipeline){latency=2}
      mask help:
      | An explicitly laid-out delay line to avoid mapping to SRL16s
      | for use in pipelining to help achieve timing closure.
      mask init:
      | pipeline_init(gcb,'latency',latency);
      settings: AttributesFormatString=Latency = %<latency>
      mask Display:
      | port_label('input', 1, 'd');
      | port_label('output', 1, 'q');
      | disp(['Z^-', num2str(latency)]);
  pipeline38 : Subsystem  AncestorBlock=casper_library_delays/pipeline  mask(pipeline){latency=2}
      mask help:
      | An explicitly laid-out delay line to avoid mapping to SRL16s
      | for use in pipelining to help achieve timing closure.
      mask init:
      | pipeline_init(gcb,'latency',latency);
      settings: AttributesFormatString=Latency = %<latency>
      mask Display:
      | port_label('input', 1, 'd');
      | port_label('output', 1, 'q');
      | disp(['Z^-', num2str(latency)]);
  pipeline39 : Subsystem  AncestorBlock=casper_library_delays/pipeline  mask(pipeline){latency=2}
      mask help:
      | An explicitly laid-out delay line to avoid mapping to SRL16s
      | for use in pipelining to help achieve timing closure.
      mask init:
      | pipeline_init(gcb,'latency',latency);
      settings: AttributesFormatString=Latency = %<latency>
      mask Display:
      | port_label('input', 1, 'd');
      | port_label('output', 1, 'q');
      | disp(['Z^-', num2str(latency)]);
  pipeline4 : Subsystem  AncestorBlock=casper_library_delays/pipeline  mask(pipeline){latency=2}
      mask help:
      | An explicitly laid-out delay line to avoid mapping to SRL16s
      | for use in pipelining to help achieve timing closure.
      mask init:
      | pipeline_init(gcb,'latency',latency);
      settings: AttributesFormatString=Latency = %<latency>
      mask Display:
      | port_label('input', 1, 'd');
      | port_label('output', 1, 'q');
      | disp(['Z^-', num2str(latency)]);
  pipeline40 : Subsystem  AncestorBlock=casper_library_delays/pipeline  mask(pipeline){latency=1}
      mask help:
      | An explicitly laid-out delay line to avoid mapping to SRL16s
      | for use in pipelining to help achieve timing closure.
      mask init:
      | pipeline_init(gcb,'latency',latency);
      settings: AttributesFormatString=Latency = %<latency>
      mask Display:
      | port_label('input', 1, 'd');
      | port_label('output', 1, 'q');
      | disp(['Z^-', num2str(latency)]);
  pipeline41 : Subsystem  AncestorBlock=casper_library_delays/pipeline  mask(pipeline){latency=1}
      mask help:
      | An explicitly laid-out delay line to avoid mapping to SRL16s
      | for use in pipelining to help achieve timing closure.
      mask init:
      | pipeline_init(gcb,'latency',latency);
      settings: AttributesFormatString=Latency = %<latency>
      mask Display:
      | port_label('input', 1, 'd');
      | port_label('output', 1, 'q');
      | disp(['Z^-', num2str(latency)]);
  pipeline42 : Subsystem  AncestorBlock=casper_library_delays/pipeline  mask(pipeline){latency=2}
      mask help:
      | An explicitly laid-out delay line to avoid mapping to SRL16s
      | for use in pipelining to help achieve timing closure.
      mask init:
      | pipeline_init(gcb,'latency',latency);
      settings: AttributesFormatString=Latency = %<latency>
      mask Display:
      | port_label('input', 1, 'd');
      | port_label('output', 1, 'q');
      | disp(['Z^-', num2str(latency)]);
  pipeline43 : Subsystem  AncestorBlock=casper_library_delays/pipeline  mask(pipeline){latency=2}
      mask help:
      | An explicitly laid-out delay line to avoid mapping to SRL16s
      | for use in pipelining to help achieve timing closure.
      mask init:
      | pipeline_init(gcb,'latency',latency);
      settings: AttributesFormatString=Latency = %<latency>
      mask Display:
      | port_label('input', 1, 'd');
      | port_label('output', 1, 'q');
      | disp(['Z^-', num2str(latency)]);
  pipeline44 : Subsystem  AncestorBlock=casper_library_delays/pipeline  mask(pipeline){latency=2}
      mask help:
      | An explicitly laid-out delay line to avoid mapping to SRL16s
      | for use in pipelining to help achieve timing closure.
      mask init:
      | pipeline_init(gcb,'latency',latency);
      settings: AttributesFormatString=Latency = %<latency>
      mask Display:
      | port_label('input', 1, 'd');
      | port_label('output', 1, 'q');
      | disp(['Z^-', num2str(latency)]);
  pipeline45 : Subsystem  AncestorBlock=casper_library_delays/pipeline  mask(pipeline){latency=2}
      mask help:
      | An explicitly laid-out delay line to avoid mapping to SRL16s
      | for use in pipelining to help achieve timing closure.
      mask init:
      | pipeline_init(gcb,'latency',latency);
      settings: AttributesFormatString=Latency = %<latency>
      mask Display:
      | port_label('input', 1, 'd');
      | port_label('output', 1, 'q');
      | disp(['Z^-', num2str(latency)]);
  pipeline46 : Subsystem  AncestorBlock=casper_library_delays/pipeline  mask(pipeline){latency=5}
      mask help:
      | An explicitly laid-out delay line to avoid mapping to SRL16s
      | for use in pipelining to help achieve timing closure.
      mask init:
      | pipeline_init(gcb,'latency',latency);
      settings: AttributesFormatString=Latency = %<latency>
      mask Display:
      | port_label('input', 1, 'd');
      | port_label('output', 1, 'q');
      | disp(['Z^-', num2str(latency)]);
  pipeline47 : Subsystem  AncestorBlock=casper_library_delays/pipeline  mask(pipeline){latency=5}
      mask help:
      | An explicitly laid-out delay line to avoid mapping to SRL16s
      | for use in pipelining to help achieve timing closure.
      mask init:
      | pipeline_init(gcb,'latency',latency);
      settings: AttributesFormatString=Latency = %<latency>
      mask Display:
      | port_label('input', 1, 'd');
      | port_label('output', 1, 'q');
      | disp(['Z^-', num2str(latency)]);
  pipeline48 : Subsystem  AncestorBlock=casper_library_delays/pipeline  mask(pipeline){latency=2}
      mask help:
      | An explicitly laid-out delay line to avoid mapping to SRL16s
      | for use in pipelining to help achieve timing closure.
      mask init:
      | pipeline_init(gcb,'latency',latency);
      settings: AttributesFormatString=Latency = %<latency>
      mask Display:
      | port_label('input', 1, 'd');
      | port_label('output', 1, 'q');
      | disp(['Z^-', num2str(latency)]);
  pipeline49 : Subsystem  AncestorBlock=casper_library_delays/pipeline  mask(pipeline){latency=2}
      mask help:
      | An explicitly laid-out delay line to avoid mapping to SRL16s
      | for use in pipelining to help achieve timing closure.
      mask init:
      | pipeline_init(gcb,'latency',latency);
      settings: AttributesFormatString=Latency = %<latency>
      mask Display:
      | port_label('input', 1, 'd');
      | port_label('output', 1, 'q');
      | disp(['Z^-', num2str(latency)]);
  pipeline5 : Subsystem  AncestorBlock=casper_library_delays/pipeline  mask(pipeline){latency=2}
      mask help:
      | An explicitly laid-out delay line to avoid mapping to SRL16s
      | for use in pipelining to help achieve timing closure.
      mask init:
      | pipeline_init(gcb,'latency',latency);
      settings: AttributesFormatString=Latency = %<latency>
      mask Display:
      | port_label('input', 1, 'd');
      | port_label('output', 1, 'q');
      | disp(['Z^-', num2str(latency)]);
  pipeline50 : Subsystem  AncestorBlock=casper_library_delays/pipeline  mask(pipeline){latency=2}
      mask help:
      | An explicitly laid-out delay line to avoid mapping to SRL16s
      | for use in pipelining to help achieve timing closure.
      mask init:
      | pipeline_init(gcb,'latency',latency);
      settings: AttributesFormatString=Latency = %<latency>
      mask Display:
      | port_label('input', 1, 'd');
      | port_label('output', 1, 'q');
      | disp(['Z^-', num2str(latency)]);
  pipeline51 : Subsystem  AncestorBlock=casper_library_delays/pipeline  mask(pipeline){latency=2}
      mask help:
      | An explicitly laid-out delay line to avoid mapping to SRL16s
      | for use in pipelining to help achieve timing closure.
      mask init:
      | pipeline_init(gcb,'latency',latency);
      settings: AttributesFormatString=Latency = %<latency>
      mask Display:
      | port_label('input', 1, 'd');
      | port_label('output', 1, 'q');
      | disp(['Z^-', num2str(latency)]);
  pipeline6 : Subsystem  AncestorBlock=casper_library_delays/pipeline  mask(pipeline){latency=5}
      mask help:
      | An explicitly laid-out delay line to avoid mapping to SRL16s
      | for use in pipelining to help achieve timing closure.
      mask init:
      | pipeline_init(gcb,'latency',latency);
      settings: AttributesFormatString=Latency = %<latency>
      mask Display:
      | port_label('input', 1, 'd');
      | port_label('output', 1, 'q');
      | disp(['Z^-', num2str(latency)]);
  pipeline67 : Subsystem  AncestorBlock=casper_library_delays/pipeline  mask(pipeline){latency=2}
      mask help:
      | An explicitly laid-out delay line to avoid mapping to SRL16s
      | for use in pipelining to help achieve timing closure.
      mask init:
      | pipeline_init(gcb,'latency',latency);
      settings: AttributesFormatString=Latency = %<latency>
      mask Display:
      | port_label('input', 1, 'd');
      | port_label('output', 1, 'q');
      | disp(['Z^-', num2str(latency)]);
  pipeline68 : Subsystem  AncestorBlock=casper_library_delays/pipeline  mask(pipeline){latency=2}
      mask help:
      | An explicitly laid-out delay line to avoid mapping to SRL16s
      | for use in pipelining to help achieve timing closure.
      mask init:
      | pipeline_init(gcb,'latency',latency);
      settings: AttributesFormatString=Latency = %<latency>
      mask Display:
      | port_label('input', 1, 'd');
      | port_label('output', 1, 'q');
      | disp(['Z^-', num2str(latency)]);
  pipeline69 : Subsystem  AncestorBlock=casper_library_delays/pipeline  mask(pipeline){latency=2}
      mask help:
      | An explicitly laid-out delay line to avoid mapping to SRL16s
      | for use in pipelining to help achieve timing closure.
      mask init:
      | pipeline_init(gcb,'latency',latency);
      settings: AttributesFormatString=Latency = %<latency>
      mask Display:
      | port_label('input', 1, 'd');
      | port_label('output', 1, 'q');
      | disp(['Z^-', num2str(latency)]);
  pipeline7 : Subsystem  AncestorBlock=casper_library_delays/pipeline  mask(pipeline){latency=5}
      mask help:
      | An explicitly laid-out delay line to avoid mapping to SRL16s
      | for use in pipelining to help achieve timing closure.
      mask init:
      | pipeline_init(gcb,'latency',latency);
      settings: AttributesFormatString=Latency = %<latency>
      mask Display:
      | port_label('input', 1, 'd');
      | port_label('output', 1, 'q');
      | disp(['Z^-', num2str(latency)]);
  pipeline70 : Subsystem  AncestorBlock=casper_library_delays/pipeline  mask(pipeline){latency=2}
      mask help:
      | An explicitly laid-out delay line to avoid mapping to SRL16s
      | for use in pipelining to help achieve timing closure.
      mask init:
      | pipeline_init(gcb,'latency',latency);
      settings: AttributesFormatString=Latency = %<latency>
      mask Display:
      | port_label('input', 1, 'd');
      | port_label('output', 1, 'q');
      | disp(['Z^-', num2str(latency)]);
  pipeline79 : Subsystem  AncestorBlock=casper_library_delays/pipeline  mask(pipeline){latency=2}
      mask help:
      | An explicitly laid-out delay line to avoid mapping to SRL16s
      | for use in pipelining to help achieve timing closure.
      mask init:
      | pipeline_init(gcb,'latency',latency);
      settings: AttributesFormatString=Latency = %<latency>
      mask Display:
      | port_label('input', 1, 'd');
      | port_label('output', 1, 'q');
      | disp(['Z^-', num2str(latency)]);
  pipeline8 : Subsystem  AncestorBlock=casper_library_delays/pipeline  mask(pipeline){latency=5}
      mask help:
      | An explicitly laid-out delay line to avoid mapping to SRL16s
      | for use in pipelining to help achieve timing closure.
      mask init:
      | pipeline_init(gcb,'latency',latency);
      settings: AttributesFormatString=Latency = %<latency>
      mask Display:
      | port_label('input', 1, 'd');
      | port_label('output', 1, 'q');
      | disp(['Z^-', num2str(latency)]);
  pipeline80 : Subsystem  AncestorBlock=casper_library_delays/pipeline  mask(pipeline){latency=2}
      mask help:
      | An explicitly laid-out delay line to avoid mapping to SRL16s
      | for use in pipelining to help achieve timing closure.
      mask init:
      | pipeline_init(gcb,'latency',latency);
      settings: AttributesFormatString=Latency = %<latency>
      mask Display:
      | port_label('input', 1, 'd');
      | port_label('output', 1, 'q');
      | disp(['Z^-', num2str(latency)]);
  pipeline81 : Subsystem  AncestorBlock=casper_library_delays/pipeline  mask(pipeline){latency=2}
      mask help:
      | An explicitly laid-out delay line to avoid mapping to SRL16s
      | for use in pipelining to help achieve timing closure.
      mask init:
      | pipeline_init(gcb,'latency',latency);
      settings: AttributesFormatString=Latency = %<latency>
      mask Display:
      | port_label('input', 1, 'd');
      | port_label('output', 1, 'q');
      | disp(['Z^-', num2str(latency)]);
  pipeline82 : Subsystem  AncestorBlock=casper_library_delays/pipeline  mask(pipeline){latency=2}
      mask help:
      | An explicitly laid-out delay line to avoid mapping to SRL16s
      | for use in pipelining to help achieve timing closure.
      mask init:
      | pipeline_init(gcb,'latency',latency);
      settings: AttributesFormatString=Latency = %<latency>
      mask Display:
      | port_label('input', 1, 'd');
      | port_label('output', 1, 'q');
      | disp(['Z^-', num2str(latency)]);
  pipeline84 : Subsystem  AncestorBlock=casper_library_delays/pipeline  mask(pipeline){latency=2}
      mask help:
      | An explicitly laid-out delay line to avoid mapping to SRL16s
      | for use in pipelining to help achieve timing closure.
      mask init:
      | pipeline_init(gcb,'latency',latency);
      settings: AttributesFormatString=Latency = %<latency>
      mask Display:
      | port_label('input', 1, 'd');
      | port_label('output', 1, 'q');
      | disp(['Z^-', num2str(latency)]);
  pipeline85 : Subsystem  AncestorBlock=casper_library_delays/pipeline  mask(pipeline){latency=2}
      mask help:
      | An explicitly laid-out delay line to avoid mapping to SRL16s
      | for use in pipelining to help achieve timing closure.
      mask init:
      | pipeline_init(gcb,'latency',latency);
      settings: AttributesFormatString=Latency = %<latency>
      mask Display:
      | port_label('input', 1, 'd');
      | port_label('output', 1, 'q');
      | disp(['Z^-', num2str(latency)]);
  pipeline86 : Subsystem  AncestorBlock=casper_library_delays/pipeline  mask(pipeline){latency=2}
      mask help:
      | An explicitly laid-out delay line to avoid mapping to SRL16s
      | for use in pipelining to help achieve timing closure.
      mask init:
      | pipeline_init(gcb,'latency',latency);
      settings: AttributesFormatString=Latency = %<latency>
      mask Display:
      | port_label('input', 1, 'd');
      | port_label('output', 1, 'q');
      | disp(['Z^-', num2str(latency)]);
  pipeline87 : Subsystem  AncestorBlock=casper_library_delays/pipeline  mask(pipeline){latency=2}
      mask help:
      | An explicitly laid-out delay line to avoid mapping to SRL16s
      | for use in pipelining to help achieve timing closure.
      mask init:
      | pipeline_init(gcb,'latency',latency);
      settings: AttributesFormatString=Latency = %<latency>
      mask Display:
      | port_label('input', 1, 'd');
      | port_label('output', 1, 'q');
      | disp(['Z^-', num2str(latency)]);
  pipeline88 : Subsystem  AncestorBlock=casper_library_delays/pipeline  mask(pipeline){latency=2}
      mask help:
      | An explicitly laid-out delay line to avoid mapping to SRL16s
      | for use in pipelining to help achieve timing closure.
      mask init:
      | pipeline_init(gcb,'latency',latency);
      settings: AttributesFormatString=Latency = %<latency>
      mask Display:
      | port_label('input', 1, 'd');
      | port_label('output', 1, 'q');
      | disp(['Z^-', num2str(latency)]);
  pipeline89 : Subsystem  AncestorBlock=casper_library_delays/pipeline  mask(pipeline){latency=2}
      mask help:
      | An explicitly laid-out delay line to avoid mapping to SRL16s
      | for use in pipelining to help achieve timing closure.
      mask init:
      | pipeline_init(gcb,'latency',latency);
      settings: AttributesFormatString=Latency = %<latency>
      mask Display:
      | port_label('input', 1, 'd');
      | port_label('output', 1, 'q');
      | disp(['Z^-', num2str(latency)]);
  pipeline9 : Subsystem  AncestorBlock=casper_library_delays/pipeline  mask(pipeline){latency=5}
      mask help:
      | An explicitly laid-out delay line to avoid mapping to SRL16s
      | for use in pipelining to help achieve timing closure.
      mask init:
      | pipeline_init(gcb,'latency',latency);
      settings: AttributesFormatString=Latency = %<latency>
      mask Display:
      | port_label('input', 1, 'd');
      | port_label('output', 1, 'q');
      | disp(['Z^-', num2str(latency)]);
  pipeline90 : Subsystem  AncestorBlock=casper_library_delays/pipeline  mask(pipeline){latency=2}
      mask help:
      | An explicitly laid-out delay line to avoid mapping to SRL16s
      | for use in pipelining to help achieve timing closure.
      mask init:
      | pipeline_init(gcb,'latency',latency);
      settings: AttributesFormatString=Latency = %<latency>
      mask Display:
      | port_label('input', 1, 'd');
      | port_label('output', 1, 'q');
      | disp(['Z^-', num2str(latency)]);
  pipeline91 : Subsystem  AncestorBlock=casper_library_delays/pipeline  mask(pipeline){latency=2}
      mask help:
      | An explicitly laid-out delay line to avoid mapping to SRL16s
      | for use in pipelining to help achieve timing closure.
      mask init:
      | pipeline_init(gcb,'latency',latency);
      settings: AttributesFormatString=Latency = %<latency>
      mask Display:
      | port_label('input', 1, 'd');
      | port_label('output', 1, 'q');
      | disp(['Z^-', num2str(latency)]);
  register_change_detect : Subsystem
  ss_fft : Subsystem  Tag=casper:bitsnap  AncestorBlock=casper_library_scopes/bitfield_snapshot  mask(bitsnap){io_names=[fft_ch fft_re fft_im fft_dv fft_sync fft_of conf_trdy], io_widths=[10 18 18 1 1 1 1], io_bps=[0 17 17 0 0 0 0], io_types=[0 1 1 2 2 2 2], show_format=on, snap_storage=bram, snap_dram_dimm=2, snap_dram_clock=250, snap_nsamples=10, snap_data_width=128, snap_offset=off, snap_circap=off, snap_value=off, snap_ext_arm=off, snap_ext_circ=off, snap_provide_outputs=on, snap_use_dsp48=on, snap_delay=2, extra_names=timestamp, extra_widths=32, extra_bps=0, extra_types=0}
      mask prompts: io_names "Names [msb...lsb]"; io_widths "Bitwidths [msb...lsb]"; io_bps "Binary pts [msb...lsb]"; io_types "Data types [msb...lsb], ufix=0, fix=1, bool=2"; show_format "Print format string?"; snap_storage "Storage medium"; snap_dram_dimm "DRAM dimm"; snap_dram_clock "DRAM clock rate"; snap_nsamples "Number of Samples (2^?)"; snap_data_width "Data width"; snap_offset "Start delay support"; snap_circap "Circular capture support"; snap_value "Extra value capture support"; snap_ext_arm "External arm support"; snap_ext_circ "External circular capture support"; snap_provide_outputs "Provide outputs"; snap_use_dsp48 "Use DSP48s to implement counters"; snap_delay "Pre-snapshot delay"; extra_names "Names [msb...lsb]"; extra_widths "Widths [msb...lsb]"; extra_bps "Binary pts [msb...lsb]"; extra_types "Data types [msb...lsb], ufix=0, fix=1, bool=2"
      mask help:
      | A wrapped snapshot block. Allows specification of inputs to a snapblock word so the toolflow can automatically set up the scope.
      | See documentation for snapshot for explanation of parameters.
      mask init:
      | bitsnap_init(gcb);
      settings: AttributesFormatString=|
      | snap(7):uf10.0,f18.17,f18.17,b,b,b,b = 50 bits\n128 wide, 1024 deep
      | debugID: 20819516
      mask TypeOptions snap_storage: bram | dram
      mask Callback snap_storage: bitsnap_callback();
      mask TypeOptions snap_dram_dimm: 1 | 2 | 3 | 4
      mask TypeOptions snap_dram_clock: 200 | 250 | 266 | 300 | 333
      mask TypeOptions snap_data_width: 8 | 16 | 32 | 64 | 128
      mask Callback snap_value: bitsnap_callback();
      mask Callback snap_ext_arm: bitsnap_callback();
      mask Callback snap_ext_circ: bitsnap_callback();
      mask Callback snap_provide_outputs: bitsnap_callback();
  ss_fir_out : Subsystem  Tag=casper:bitsnap  AncestorBlock=casper_library_scopes/bitfield_snapshot  mask(bitsnap){io_names=[fir_re fir_im sync tlast dv trig trig_time], io_widths=[18 18 1 1 1 1 48], io_bps=[17 17 0 0 0 0 0], io_types=[1 1 2 2 2 2 0], show_format=on, snap_storage=bram, snap_dram_dimm=2, snap_dram_clock=250, snap_nsamples=10, snap_data_width=128, snap_offset=off, snap_circap=off, snap_value=off, snap_ext_arm=off, snap_ext_circ=off, snap_provide_outputs=on, snap_use_dsp48=on, snap_delay=2, extra_names=timestamp, extra_widths=32, extra_bps=0, extra_types=0}
      mask prompts: io_names "Names [msb...lsb]"; io_widths "Bitwidths [msb...lsb]"; io_bps "Binary pts [msb...lsb]"; io_types "Data types [msb...lsb], ufix=0, fix=1, bool=2"; show_format "Print format string?"; snap_storage "Storage medium"; snap_dram_dimm "DRAM dimm"; snap_dram_clock "DRAM clock rate"; snap_nsamples "Number of Samples (2^?)"; snap_data_width "Data width"; snap_offset "Start delay support"; snap_circap "Circular capture support"; snap_value "Extra value capture support"; snap_ext_arm "External arm support"; snap_ext_circ "External circular capture support"; snap_provide_outputs "Provide outputs"; snap_use_dsp48 "Use DSP48s to implement counters"; snap_delay "Pre-snapshot delay"; extra_names "Names [msb...lsb]"; extra_widths "Widths [msb...lsb]"; extra_bps "Binary pts [msb...lsb]"; extra_types "Data types [msb...lsb], ufix=0, fix=1, bool=2"
      mask help:
      | A wrapped snapshot block. Allows specification of inputs to a snapblock word so the toolflow can automatically set up the scope.
      | See documentation for snapshot for explanation of parameters.
      mask init:
      | bitsnap_init(gcb);
      settings: AttributesFormatString=|
      | snap(7):f18.17,f18.17,b,b,b,b,uf48.0 = 88 bits\n128 wide, 1024 deep
      | debugID: 62424594
      mask TypeOptions snap_storage: bram | dram
      mask Callback snap_storage: bitsnap_callback();
      mask TypeOptions snap_dram_dimm: 1 | 2 | 3 | 4
      mask TypeOptions snap_dram_clock: 200 | 250 | 266 | 300 | 333
      mask TypeOptions snap_data_width: 8 | 16 | 32 | 64 | 128
      mask Callback snap_value: bitsnap_callback();
      mask Callback snap_ext_arm: bitsnap_callback();
      mask Callback snap_ext_circ: bitsnap_callback();
      mask Callback snap_provide_outputs: bitsnap_callback();
  ss_nb : Subsystem  Tag=casper:bitsnap  AncestorBlock=casper_library_scopes/bitfield_snapshot  mask(bitsnap){io_names=[r0 i0 r1 i1 sync dv sync_cnt new_spec trig trig_time ch], io_widths=[18 18 18 18 1 1 4 1 1 38 10], io_bps=[17 17 17 17 0 0 0 0 0 0 0], io_types=[1 1 1 1 2 2 0 2 2 0 0], show_format=on, snap_storage=bram, snap_dram_dimm=2, snap_dram_clock=250, snap_nsamples=9, snap_data_width=128, snap_offset=off, snap_circap=off, snap_value=off, snap_ext_arm=off, snap_ext_circ=off, snap_provide_outputs=on, snap_use_dsp48=on, snap_delay=2, extra_names=timestamp, extra_widths=32, extra_bps=0, extra_types=0}
      mask prompts: io_names "Names [msb...lsb]"; io_widths "Bitwidths [msb...lsb]"; io_bps "Binary pts [msb...lsb]"; io_types "Data types [msb...lsb], ufix=0, fix=1, bool=2"; show_format "Print format string?"; snap_storage "Storage medium"; snap_dram_dimm "DRAM dimm"; snap_dram_clock "DRAM clock rate"; snap_nsamples "Number of Samples (2^?)"; snap_data_width "Data width"; snap_offset "Start delay support"; snap_circap "Circular capture support"; snap_value "Extra value capture support"; snap_ext_arm "External arm support"; snap_ext_circ "External circular capture support"; snap_provide_outputs "Provide outputs"; snap_use_dsp48 "Use DSP48s to implement counters"; snap_delay "Pre-snapshot delay"; extra_names "Names [msb...lsb]"; extra_widths "Widths [msb...lsb]"; extra_bps "Binary pts [msb...lsb]"; extra_types "Data types [msb...lsb], ufix=0, fix=1, bool=2"
      mask help:
      | A wrapped snapshot block. Allows specification of inputs to a snapblock word so the toolflow can automatically set up the scope.
      | See documentation for snapshot for explanation of parameters.
      mask init:
      | bitsnap_init(gcb);
      settings: AttributesFormatString=|
      | snap(11):f18.17,f18.17,f18.17,f18.17,b,b,uf4.0,b,b,uf38.0,uf10.0 = 128 bits\n128 wide, 512 deep
      | debugID: 55502042
      mask TypeOptions snap_storage: bram | dram
      mask Callback snap_storage: bitsnap_callback();
      mask TypeOptions snap_dram_dimm: 1 | 2 | 3 | 4
      mask TypeOptions snap_dram_clock: 200 | 250 | 266 | 300 | 333
      mask TypeOptions snap_data_width: 8 | 16 | 32 | 64 | 128
      mask Callback snap_value: bitsnap_callback();
      mask Callback snap_ext_arm: bitsnap_callback();
      mask Callback snap_ext_circ: bitsnap_callback();
      mask Callback snap_provide_outputs: bitsnap_callback();
  ss_nb1 : Subsystem  Tag=casper:bitsnap  AncestorBlock=casper_library_scopes/bitfield_snapshot  mask(bitsnap){io_names=[r2 i2 r3 i3 sync dv sync_cnt trig trig_time], io_widths=[18 18 18 18 1 1 4 1 48], io_bps=[17 17 17 17 0 0 0 0 0], io_types=[1 1 1 1 2 2 0 2 0], show_format=on, snap_storage=bram, snap_dram_dimm=2, snap_dram_clock=250, snap_nsamples=9, snap_data_width=128, snap_offset=off, snap_circap=off, snap_value=off, snap_ext_arm=off, snap_ext_circ=off, snap_provide_outputs=on, snap_use_dsp48=on, snap_delay=2, extra_names=timestamp, extra_widths=32, extra_bps=0, extra_types=0}
      mask prompts: io_names "Names [msb...lsb]"; io_widths "Bitwidths [msb...lsb]"; io_bps "Binary pts [msb...lsb]"; io_types "Data types [msb...lsb], ufix=0, fix=1, bool=2"; show_format "Print format string?"; snap_storage "Storage medium"; snap_dram_dimm "DRAM dimm"; snap_dram_clock "DRAM clock rate"; snap_nsamples "Number of Samples (2^?)"; snap_data_width "Data width"; snap_offset "Start delay support"; snap_circap "Circular capture support"; snap_value "Extra value capture support"; snap_ext_arm "External arm support"; snap_ext_circ "External circular capture support"; snap_provide_outputs "Provide outputs"; snap_use_dsp48 "Use DSP48s to implement counters"; snap_delay "Pre-snapshot delay"; extra_names "Names [msb...lsb]"; extra_widths "Widths [msb...lsb]"; extra_bps "Binary pts [msb...lsb]"; extra_types "Data types [msb...lsb], ufix=0, fix=1, bool=2"
      mask help:
      | A wrapped snapshot block. Allows specification of inputs to a snapblock word so the toolflow can automatically set up the scope.
      | See documentation for snapshot for explanation of parameters.
      mask init:
      | bitsnap_init(gcb);
      settings: AttributesFormatString=|
      | snap(9):f18.17,f18.17,f18.17,f18.17,b,b,uf4.0,b,uf48.0 = 127 bits\n128 wide, 512 deep
      | debugID: 109944915
      mask TypeOptions snap_storage: bram | dram
      mask Callback snap_storage: bitsnap_callback();
      mask TypeOptions snap_dram_dimm: 1 | 2 | 3 | 4
      mask TypeOptions snap_dram_clock: 200 | 250 | 266 | 300 | 333
      mask TypeOptions snap_data_width: 8 | 16 | 32 | 64 | 128
      mask Callback snap_value: bitsnap_callback();
      mask Callback snap_ext_arm: bitsnap_callback();
      mask Callback snap_ext_circ: bitsnap_callback();
      mask Callback snap_provide_outputs: bitsnap_callback();
  ss_nb_sync : Subsystem  Tag=casper:bitsnap  AncestorBlock=casper_library_scopes/bitfield_snapshot  mask(bitsnap){io_names=[re im sync dv re_ord_ch sync_cnt trig trig_time reord_mux_sel reg_ch], io_widths=[18 18 1 1 10 fft_stages 1 48 1 10], io_bps=[17 17 0 0 0 0 0 0 0 0], io_types=[1 1 2 2 0 0 2 0 2 0], show_format=on, snap_storage=bram, snap_dram_dimm=2, snap_dram_clock=250, snap_nsamples=10, snap_data_width=128, snap_offset=off, snap_circap=off, snap_value=off, snap_ext_arm=off, snap_ext_circ=off, snap_provide_outputs=on, snap_use_dsp48=on, snap_delay=2, extra_names=timestamp, extra_widths=32, extra_bps=0, extra_types=0}
      mask prompts: io_names "Names [msb...lsb]"; io_widths "Bitwidths [msb...lsb]"; io_bps "Binary pts [msb...lsb]"; io_types "Data types [msb...lsb], ufix=0, fix=1, bool=2"; show_format "Print format string?"; snap_storage "Storage medium"; snap_dram_dimm "DRAM dimm"; snap_dram_clock "DRAM clock rate"; snap_nsamples "Number of Samples (2^?)"; snap_data_width "Data width"; snap_offset "Start delay support"; snap_circap "Circular capture support"; snap_value "Extra value capture support"; snap_ext_arm "External arm support"; snap_ext_circ "External circular capture support"; snap_provide_outputs "Provide outputs"; snap_use_dsp48 "Use DSP48s to implement counters"; snap_delay "Pre-snapshot delay"; extra_names "Names [msb...lsb]"; extra_widths "Widths [msb...lsb]"; extra_bps "Binary pts [msb...lsb]"; extra_types "Data types [msb...lsb], ufix=0, fix=1, bool=2"
      mask help:
      | A wrapped snapshot block. Allows specification of inputs to a snapblock word so the toolflow can automatically set up the scope.
      | See documentation for snapshot for explanation of parameters.
      mask init:
      | bitsnap_init(gcb);
      settings: AttributesFormatString=|
      | snap(10):f18.17,f18.17,b,b,uf10.0,uf11.0,b,uf48.0,b,uf10.0 = 119 bits\n128 wide, 1024 deep
      | debugID: 85027306
      mask TypeOptions snap_storage: bram | dram
      mask Callback snap_storage: bitsnap_callback();
      mask TypeOptions snap_dram_dimm: 1 | 2 | 3 | 4
      mask TypeOptions snap_dram_clock: 200 | 250 | 266 | 300 | 333
      mask TypeOptions snap_data_width: 8 | 16 | 32 | 64 | 128
      mask Callback snap_value: bitsnap_callback();
      mask Callback snap_ext_arm: bitsnap_callback();
      mask Callback snap_ext_circ: bitsnap_callback();
      mask Callback snap_provide_outputs: bitsnap_callback();
  ss_time_trig_fir : Subsystem
  ss_time_trig_nb : Subsystem
  ss_time_trig_syncgen : Subsystem
  sync_out : Outport
  dv_out : Outport  Port=2
  pol0_out : Outport  Port=3
  pol1_out : Outport  Port=4
  pfb_of : Outport  Port=5
  tag scope: capture_now=global, current_channel=global, data_pol0=global, fft_ch0=global, fft_ch1=global, fft_conf_tready_p0=global, fft_config_reload=global, fft_dv0=global, fft_dv1=global, fft_dvalid=global, fft_pol0_of=global, fft_pol1_of=global, fft_sync0=global, fft_sync=global, fft_sync_count=global, fft_tready_p0=global, fir_data_tlast=global, fir_dvalid_pol0=global, fir_pol0=global, fir_sync=global, reg_channel=global, reord_channel=global, reord_dv=global, reord_mux_sel=global, reord_mux_sel_ext=global, reord_pol0=global, reord_pol1=global, reord_sync=global
  wires:
  pfb_fir_generic/2(pol0_out0) -> pipeline18/1(d)
  pfb_fir_generic1/2(pol0_out0) -> pipeline20/1(d)
  pfb_fir_generic/1(sync_out) -> pipeline17/1(d)
  pfb_fir_generic1/1(sync_out) -> Terminator5/1
  Reinterpret2/1 -> Concat3/1
  Reinterpret3/1 -> Concat3/2
  Concat3/1 -> [data_pol1]
  pol1/1 -> pfb_fir_generic1/2(pol0_in0)
  pipeline20/1(q) -> Delay37/1
  Gateway Out21/1 -> To Workspace21/1
  bus_expand1/1(msb_out8) -> Gateway Out21/1
  Gateway Out23/1 -> To Workspace23/1
  bus_expand1/2(out7) -> Gateway Out23/1
  Gateway Out24/1 -> To Workspace24/1
  bus_expand1/3(out6) -> Gateway Out24/1
  Gateway Out25/1 -> To Workspace27/1
  bus_expand1/4(out5) -> Gateway Out25/1
  Gateway Out28/1 -> To Workspace25/1
  bus_expand1/5(out4) -> Gateway Out28/1
  Gateway Out29/1 -> To Workspace28/1
  bus_expand1/6(out3) -> Gateway Out29/1
  Gateway Out30/1 -> To Workspace26/1
  bus_expand1/7(out2) -> Gateway Out30/1
  Gateway Out31/1 -> To Workspace29/1
  bus_expand1/8(lsb_out1) -> Gateway Out31/1
  Gateway Out6/1 -> To Workspace6/1
  Gateway Out1/1 -> To Workspace1/1
  Gateway Out9/1 -> To Workspace9/1
  Gateway Out36/1 -> To Workspace36/1
  Gateway Out39/1 -> To Workspace39/1
  Delay13/1 -> Reinterpret3/1
  Delay11/1 -> Reinterpret2/1
  pfb_fir_generic/3(dvalid) -> pipeline19/1(d)
  pfb_fir_generic1/3(dvalid) -> pipeline21/1(d)
  Counter1/1 -> pipeline81/1(d), pipeline69/1(d)
  pipeline67/1(q) -> ss_nb/5(in_sync)
  pipeline68/1(q) -> ss_nb/6(in_dv)
  pipeline69/1(q) -> ss_nb/7(in_sync_cnt)
  pipeline70/1(q) -> ss_nb/9(in_trig)
  pipeline39/1(q) -> ss_nb/10(in_trig_time)
  sync/1 -> pfb_fir_generic1/1(sync), Gateway Out9/1, pfb_fir_generic/1(sync)
  [fir_dvalid_pol0] -> pipeline9/1(d), pipeline6/1(d)
  pipeline9/1(q) -> ss_fir_out/8(we)
  [fir_sync] -> pipeline7/1(d)
  Relational4/1 -> Delay68/1
  Counter3/1 -> Relational4/1, Gateway Out53/1
  Constant9/1 -> Relational4/2
  pipeline7/1(q) -> ss_fir_out/3(in_sync)
  pipeline6/1(q) -> ss_fir_out/5(in_dv)
  bus_expand2/1(msb_out8) -> pipeline87/1(d)
  bus_expand2/2(out7) -> pipeline86/1(d)
  bus_expand2/3(out6) -> pipeline85/1(d)
  bus_expand2/4(out5) -> pipeline84/1(d)
  pipeline84/1(q) -> ss_nb/4(in_i1)
  pipeline85/1(q) -> ss_nb/3(in_r1)
  pipeline86/1(q) -> ss_nb/2(in_i0)
  pipeline87/1(q) -> ss_nb/1(in_r0)
  pipeline79/1(q) -> ss_nb1/5(in_sync)
  pipeline80/1(q) -> ss_nb1/6(in_dv)
  pipeline81/1(q) -> ss_nb1/7(in_sync_cnt)
  pipeline82/1(q) -> ss_nb1/8(in_trig)
  pipeline38/1(q) -> ss_nb1/9(in_trig_time)
  bus_expand2/5(out4) -> pipeline91/1(d)
  bus_expand2/6(out3) -> pipeline90/1(d)
  bus_expand2/7(out2) -> pipeline89/1(d)
  bus_expand2/8(lsb_out1) -> pipeline88/1(d)
  dvalid/1 -> pfb_fir_generic1/3(en), Gateway Out36/1, pfb_fir_generic/3(en)
  [fft_ch0] -> pipeline126/1(d)
  [fft_dv0] -> pipeline4/1(d), pipeline129/1(d)
  pipeline126/1(q) -> ss_fft/1(in_fft_ch)
  pipeline127/1(q) -> ss_fft/2(in_fft_re)
  pipeline128/1(q) -> ss_fft/3(in_fft_im)
  pipeline129/1(q) -> ss_fft/4(in_fft_dv)
  [fft_sync0] -> pipeline13/1(d), pipeline131/1(d)
  [fft_pol0_of] -> pipeline132/1(d)
  pipeline132/1(q) -> ss_fft/6(in_fft_of)
  pipeline131/1(q) -> ss_fft/5(in_fft_sync)
  Gateway Out70/1 -> To Workspace69/1
  Gateway Out71/1 -> To Workspace70/1
  [fft_re_pol0] -> Gateway Out70/1
  [fft_im_pol0] -> Gateway Out71/1
  pol0/1 -> bus_expand14/1(bus_in), pfb_fir_generic/2(pol0_in0)
  [fft_re_pol0] -> pipeline127/1(d)
  [fft_im_pol0] -> pipeline128/1(d)
  pipeline88/1(q) -> ss_nb1/4(in_i3)
  pipeline89/1(q) -> ss_nb1/3(in_r3)
  pipeline90/1(q) -> ss_nb1/2(in_i2)
  pipeline91/1(q) -> ss_nb1/1(in_r2)
  pipeline42/1(q) -> ss_nb/8(in_new_spec)
  [new_spec] -> pipeline42/1(d)
  fft_shift/1 -> [fft_shift]
  Constant2/1 -> Mux3/2
  [fft_dv0] -> Mux3/1
  Mux3/1 -> [fft_re_pol0]
  Constant1/1 -> Mux4/2
  Mux4/1 -> [fft_im_pol0]
  [fft_re_pol0_int] -> Mux3/3
  [fft_im_pol0_int] -> Mux4/3
  [fft_dv0] -> Mux4/1
  Delay6/1 -> [fir_dvalid_pol0], Gateway Out1/1
  pipeline17/1(q) -> Delay89/1, Counter3/1
  Delay37/1 -> [fir_pol1]
  Delay38/1 -> [fir_dvalid_pol1]
  [fir_data_tlast] -> pipeline25/1(d)
  pipeline25/1(q) -> ss_fir_out/4(in_tlast)
  pipeline18/1(q) -> Delay15/1
  pipeline21/1(q) -> Delay38/1
  Delay15/1 -> [fir_pol0]
  [sync_out] -> pipeline79/1(d), pipeline67/1(d)
  [cnt_rst] -> pipeline230/1(d)
  Counter12/1 -> fir_sync_cnt/1(out_reg)
  pipeline229/1(q) -> Counter12/2
  pipeline230/1(q) -> Counter12/1
  pipeline19/1(q) -> Delay6/1, Counter3/2
  pipeline4/1(q) -> ss_fft/8(we)
  [reord_pol0] -> bus_expand8/1(bus_in)
  [ts_ss_lock] -> Mux5/1
  Mux5/1 -> edge_detect4/1(in)
  [arm_ts_ss_rst] -> ss_time_trig_syncgen/2(rst)
  [arm_ts_ss_lock] -> ss_time_trig_syncgen/3(arm)
  ss_time_trig_syncgen/1(trig) -> Mux5/3
  [ss_trig_time_in] -> ss_time_trig_syncgen/4(trig_time_in)
  [time80_48] -> ss_time_trig_syncgen/1(current_time)
  edge_detect4/1(out) -> pipeline35/1(d), pipeline26/1(d)
  ss_time_trig_syncgen/2(trig_time) -> pipeline36/1(d)
  bus_expand8/1(msb_out2) -> pipeline29/1(d)
  bus_expand8/2(lsb_out1) -> pipeline30/1(d)
  [reord_sync] -> pipeline31/1(d)
  [reord_dv] -> pipeline15/1(d), pipeline32/1(d)
  [fft_sync_count] -> pipeline34/1(d)
  [reord_sync] -> Mux5/2
  pipeline29/1(q) -> ss_nb_sync/1(in_re)
  pipeline30/1(q) -> ss_nb_sync/2(in_im)
  pipeline31/1(q) -> ss_nb_sync/3(in_sync)
  pipeline32/1(q) -> ss_nb_sync/4(in_dv)
  pipeline34/1(q) -> ss_nb_sync/6(in_sync_cnt)
  pipeline35/1(q) -> ss_nb_sync/7(in_trig)
  pipeline36/1(q) -> ss_nb_sync/8(in_trig_time)
  pipeline15/1(q) -> ss_nb_sync/11(we)
  [ts_ss_lock] -> Mux6/1
  Mux6/1 -> edge_detect6/1(in)
  [arm_ts_ss_rst] -> ss_time_trig_nb/2(rst)
  [arm_ts_ss_lock] -> ss_time_trig_nb/3(arm)
  ss_time_trig_nb/1(trig) -> Mux6/3
  [ss_trig_time_in] -> ss_time_trig_nb/4(trig_time_in)
  [time80_48] -> ss_time_trig_nb/1(current_time)
  [sync_out] -> Mux6/2
  pipeline28/1(q) -> ss_nb1/10(we)
  pipeline37/1(q) -> ss_nb/12(we)
  ss_time_trig_nb/2(trig_time) -> pipeline38/1(d), Slice5/1
  edge_detect6/1(out) -> pipeline40/1(d), pipeline41/1(d), pipeline82/1(d), pipeline70/1(d)
  [ts_ss_lock] -> Mux8/1
  Mux8/1 -> edge_detect5/1(in)
  ss_time_trig_fir/1(trig) -> Mux8/3
  [arm_ts_ss_rst] -> ss_time_trig_fir/2(rst)
  [arm_ts_ss_lock] -> ss_time_trig_fir/3(arm)
  [ss_trig_time_in] -> ss_time_trig_fir/4(trig_time_in)
  [time80_48] -> ss_time_trig_fir/1(current_time)
  [fir_sync] -> Mux8/2
  pipeline46/1(q) -> ss_fir_out/7(in_trig_time)
  pipeline47/1(q) -> ss_fir_out/6(in_trig)
  edge_detect5/1(out) -> pipeline10/1(d), pipeline47/1(d)
  ss_time_trig_fir/2(trig_time) -> pipeline46/1(d)
  Fast Fourier Transform 9.0 1/1 -> pipeline23/1(d)
  Fast Fourier Transform 9.0 1/2 -> pipeline117/1(d)
  pipeline117/1(q) -> [fft_tready_p0]
  pipeline110/1(q) -> [fft_ch0]
  Gateway Out66/1 -> To Workspace65/1
  Gateway Out67/1 -> To Workspace66/1
  Gateway Out72/1 -> To Workspace71/1
  [fft_dv0] -> Gateway Out67/1
  [fft_ch0] -> Gateway Out66/1
  [fft_tready_p0] -> Gateway Out72/1
  Fast Fourier Transform 9.0 1/5 -> pipeline122/1(d)
  Fast Fourier Transform 9.0 1/6 -> pipeline123/1(d)
  Fast Fourier Transform 9.0 1/8 -> pipeline110/1(d), Relational2/1
  Fast Fourier Transform 9.0 1/15 -> Terminator7/1
  Fast Fourier Transform 9.0 1/16 -> Terminator8/1
  Fast Fourier Transform 9.0 1/17 -> Terminator9/1
  [fft_shift] -> Slice/1
  [fir_data_tlast] -> Delay67/1
  pipeline123/1(q) -> [fft_re_pol0_int]
  pipeline122/1(q) -> [fft_im_pol0_int]
  Inverter1/1 -> Logical1/2, Fast Fourier Transform 9.0 1/10
  Logical11/1 -> Inverter1/1
  Gateway Out37/1 -> To Workspace37/1
  [fir_sync] -> Delay118/1, Delay97/1, Logical11/1
  [fft_sync0] -> Gateway Out37/1
  Concat/1 -> [data_pol0]
  Gateway Out34/1 -> To Workspace32/1
  Delay44/1 -> [fft_sync]
  [current_channel] -> Gateway Out34/1
  [fft_sync0] -> Delay44/1
  Delay17/1 -> [current_channel]
  Delay8/1 -> Reinterpret1/1
  Delay9/1 -> Reinterpret/1
  [data_pol0] -> bus_expand16/1(bus_in)
  Gateway Out2/1 -> To Workspace2/1
  Gateway Out5/1 -> To Workspace5/1
  Delay2/1 -> [fft_dvalid]
  [fft_im_pol0] -> Delay8/1
  [fft_re_pol0] -> Delay9/1
  [fft_dv0] -> Delay2/1
  [fft_ch0] -> Delay17/1
  [cnt_rst] -> pipeline27/1(d)
  Counter4/1 -> [fft_sync_count], fft_sync_cnt/1(out_reg)
  pipeline1/1(q) -> Counter4/2
  pipeline27/1(q) -> Counter4/1
  [fft_sync] -> pipeline1/1(d)
  [nb_dv] -> pipeline68/1(d), pipeline37/1(d), pipeline28/1(d), pipeline80/1(d)
  [pol0] -> bus_expand1/1(bus_in), bus_expand2/1(bus_in)
  Gateway Out18/1 -> To Workspace19/1
  Register11/1 -> bus_expand7/1(bus_in), Delay26/1
  Register10/1 -> Delay25/1
  Register9/1 -> Delay23/1
  Register1/1 -> bus_expand6/1(bus_in), Delay22/1
  [capture_now] -> Register1/3
  [capture_now] -> Register9/3
  [capture_now] -> Register10/3
  [capture_now] -> Register11/3
  Gateway Out7/1 -> To Workspace7/1
  Delay19/1 -> Register9/1
  Delay20/1 -> Register10/1
  Gateway Out40/1 -> To Workspace40/1
  Concat5/1 -> pipeline45/1(d)
  [reord_channel] -> Delay5/1
  lsb_1/1 -> Logical4/2
  lsb_0/1 -> Logical4/1
  Logical4/1 -> edge_detect2/1(in)
  [reord_dv] -> Delay1/1
  edge_detect2/1(out) -> [capture_now], Gateway Out40/1
  [capture_now] -> Delay10/1
  Delay10/1 -> Gateway Out61/1, Delay32/1
  Delay1/1 -> Logical4/3
  bus_expand5/1(msb_out2) -> Gateway Out46/1
  bus_expand5/2(lsb_out1) -> Gateway Out49/1
  Delay16/1 -> bus_expand5/1(bus_in), Register1/1
  Gateway Out12/1 -> To Workspace12/1
  Gateway Out13/1 -> To Workspace13/1
  bus_expand4/1(msb_out2) -> Gateway Out13/1
  Gateway Out14/1 -> To Workspace14/1
  bus_expand4/2(lsb_out1) -> Gateway Out14/1
  Gateway Out46/1 -> To Workspace45/1
  Gateway Out49/1 -> To Workspace46/1
  Delay22/1 -> Delay27/1
  Delay23/1 -> Delay28/1
  Delay25/1 -> Delay29/1
  Delay26/1 -> Delay30/1
  Delay27/1 -> Concat5/1
  Delay28/1 -> Concat5/2
  Delay29/1 -> Concat5/3
  Delay30/1 -> Concat5/4
  Delay32/1 -> Delay31/1
  Gateway Out61/1 -> To Workspace49/1
  [reord_dv] -> Delay73/1
  bus_expand6/1(msb_out2) -> To Workspace64/1
  bus_expand6/2(lsb_out1) -> To Workspace73/1
  Gateway Out65/1 -> To Workspace74/1
  bus_expand7/1(msb_out2) -> Gateway Out65/1
  Gateway Out73/1 -> To Workspace75/1
  bus_expand7/2(lsb_out1) -> Gateway Out73/1
  Delay5/1 -> Gateway Out11/1, Delay33/1, Gateway Out12/1, lsb_1/1, lsb_0/1
  Delay33/1 -> Delay34/1
  Delay34/1 -> Delay35/1
  Gateway Out83/1 -> To Workspace85/1
  Delay35/1 -> Delay39/1
  Delay31/1 -> Delay14/1
  [reord_sync] -> Delay78/1
  [reord_pol0] -> Delay74/1
  Delay41/1 -> Delay40/1
  Delay14/1 -> Delay106/1
  Delay39/1 -> Delay105/1
  Gateway Out11/1 -> To Workspace11/1
  Delay40/1 -> [sync_out]
  [sync_out] -> Gateway Out7/1, sync_out/1
  Register4/1 -> Delay57/1
  Register3/1 -> Delay56/1
  Register7/1 -> Delay54/1
  Register2/1 -> Delay53/1
  [capture_now] -> Register2/3
  [capture_now] -> Register7/3
  [capture_now] -> Register3/3
  [capture_now] -> Register4/3
  Delay51/1 -> Register7/1
  Delay52/1 -> Register3/1
  Concat1/1 -> pipeline2/1(d)
  Delay7/1 -> Register2/1
  Delay53/1 -> Delay58/1
  Delay54/1 -> Delay59/1
  Delay56/1 -> Delay60/1
  Delay57/1 -> Delay61/1
  Delay58/1 -> Concat1/1
  Delay59/1 -> Concat1/2
  Delay60/1 -> Concat1/3
  Delay61/1 -> Concat1/4
  [reord_sync] -> Delay62/1
  [reord_pol1] -> Delay76/1
  Gateway Out22/1 -> To Workspace22/1
  bus_expand9/1(msb_out2) -> Gateway Out26/1
  bus_expand9/2(lsb_out1) -> Gateway Out38/1
  Gateway Out26/1 -> To Workspace30/1
  Gateway Out38/1 -> To Workspace38/1
  Delay73/1 -> Gateway Out22/1, Delay19/2, Delay20/2, Delay16/2
  Delay74/1 -> bus_expand9/1(bus_in), bus_expand4/1(bus_in), Register11/1, Delay20/1, Delay19/1, Delay16/1
  [reord_dv] -> Delay75/1
  Delay76/1 -> Register4/1, Delay52/1, Delay51/1, Delay7/1
  Delay75/1 -> Delay51/2, Delay52/2, Delay7/2
  [pol0] -> pol0_out/1
  [pol1] -> pol1_out/1
  [nb_dv] -> Gateway Out18/1, dv_out/1
  pipeline10/1(q) -> ss_fir_out/9(trig)
  [fft_re_pol1] -> Delay11/1
  [fft_im_pol1] -> Delay13/1
  [fft_shift] -> Slice1/1
  [fir_data_tlast] -> Delay84/1
  Inverter2/1 -> Fast Fourier Transform 9.0 2/10, Logical2/2
  Logical7/1 -> Inverter2/1
  pipeline12/1(q) -> [fft_ch1]
  pipeline50/1(q) -> [fft_dv1]
  pipeline48/1(q) -> [fft_re_pol1_int]
  pipeline44/1(q) -> [fft_im_pol1_int]
  Constant7/1 -> Mux9/2
  [fft_dv1] -> Mux9/1
  Mux9/1 -> [fft_re_pol1]
  Constant6/1 -> Mux10/2
  Mux10/1 -> [fft_im_pol1]
  [fft_re_pol1_int] -> Mux9/3
  [fft_im_pol1_int] -> Mux10/3
  [fft_dv1] -> Mux10/1
  [fft_ch0] -> Relational1/1
  [fft_ch1] -> Relational1/2
  Counter5/1 -> fft_ch_err/1(out_reg)
  Relational1/1 -> Counter5/2
  pipeline14/1(q) -> Counter5/1
  [cnt_rst] -> pipeline14/1(d)
  Constant12/1 -> Fast Fourier Transform 9.0 1/8
  Delay67/1 -> Fast Fourier Transform 9.0 1/7
  Delay69/1 -> Fast Fourier Transform 9.0 1/5
  Delay70/1 -> Fast Fourier Transform 9.0 1/4
  Constant10/1 -> Fast Fourier Transform 9.0 1/3
  Constant3/1 -> Fast Fourier Transform 9.0 1/2
  [fir_dvalid_pol0] -> Logical1/1
  Slice/1 -> Register/1, Fast Fourier Transform 9.0 1/1
  Delay78/1 -> Register1/2, Register11/2, Register10/2, Register9/2
  Delay42/1 -> Delay41/1
  Delay43/1 -> Delay42/1
  Slice1/1 -> Fast Fourier Transform 9.0 2/1
  Constant13/1 -> Fast Fourier Transform 9.0 2/3
  Delay81/1 -> Fast Fourier Transform 9.0 2/4
  Delay82/1 -> Fast Fourier Transform 9.0 2/5
  Delay83/1 -> Logical2/1
  Logical2/1 -> Fast Fourier Transform 9.0 2/6
  [fir_dvalid_pol1] -> Delay83/1
  Delay84/1 -> Fast Fourier Transform 9.0 2/7
  Constant8/1 -> Fast Fourier Transform 9.0 2/9
  pipeline124/1(q) -> [fft_dv0]
  edge_detect3/1(out) -> [fft_sync0]
  edge_detect1/1(out) -> Register5/2
  Register5/1 -> edge_detect3/1(in)
  [fir_pol0] -> bus_expand10/1(bus_in)
  [fir_pol1] -> bus_expand11/1(bus_in)
  Delay62/1 -> Register7/2, Register3/2, Register4/2, Register2/2
  pipeline8/1(q) -> ss_fir_out/1(in_fir_re)
  pipeline11/1(q) -> ss_fir_out/2(in_fir_im)
  pipeline13/1(q) -> ss_fft/9(trig)
  pipeline26/1(q) -> ss_nb_sync/12(trig)
  pipeline40/1(q) -> ss_nb/13(trig)
  pipeline41/1(q) -> ss_nb1/11(trig)
  bus_expand12/1(msb_out2) -> pipeline8/1(d)
  bus_expand12/2(lsb_out1) -> pipeline11/1(d)
  [fir_pol0] -> bus_expand12/1(bus_in)
  [fir_pol0] -> bus_expand13/1(bus_in)
  Gateway Out4/1 -> To Workspace4/1
  bus_expand13/1(msb_out2) -> Gateway Out4/1
  Gateway Out8/1 -> To Workspace8/1
  bus_expand13/2(lsb_out1) -> Gateway Out8/1
  bus_expand10/2(lsb_out1) -> Delay70/1
  bus_expand10/1(msb_out2) -> Delay69/1
  bus_expand11/2(lsb_out1) -> Delay81/1
  bus_expand11/1(msb_out2) -> Delay82/1
  bus_expand14/1(msb_out2) -> Gateway Out39/1
  Gateway Out35/1 -> To Workspace35/1
  bus_expand14/2(lsb_out1) -> Gateway Out35/1
  [data_pol0] -> Delay88/1, Delay46/1
  Delay24/1 -> Delay4/1
  [fft_sync] -> Gateway Out33/1, Register12/3, Register12/1
  Gateway Out15/1 -> To Workspace15/1
  Gateway Out17/1 -> To Workspace17/1
  Gateway Out20/1 -> To Workspace20/1
  [current_channel] -> Slice2/1, Slice4/1
  Constant17/1 -> AddSub/2
  AddSub/1 -> Delay3/1
  Delay12/1 -> Single Port RAM/2
  Delay18/1 -> Single Port RAM/1, Gateway Out20/1
  Gateway Out47/1 -> To Workspace48/1
  Delay46/1 -> Delay12/1
  Delay47/1 -> Delay18/1
  Delay3/1 -> Delay99/1
  Reinterpret1/1 -> Concat/2
  Reinterpret/1 -> Concat/1
  bus_expand3/2(lsb_out1) -> Gateway Out17/1
  bus_expand3/1(msb_out2) -> Gateway Out15/1
  [reord_channel] -> pipeline33/1(d)
  Gateway Out50/1 -> To Workspace51/1
  Gateway Out51/1 -> To Workspace3/1
  Gateway Out52/1 -> To Workspace16/1
  bus_expand16/1(msb_out2) -> Gateway Out2/1
  bus_expand16/2(lsb_out1) -> Gateway Out5/1
  [fft_dvalid] -> Gateway Out51/1
  [fft_sync] -> Gateway Out52/1
  Gateway Out3/1 -> To Workspace47/1
  Delay55/1 -> Delay49/1
  Gateway Out16/1 -> To Workspace42/1
  [reord_pol0] -> bus_expand3/1(bus_in)
  [reord_channel] -> Gateway Out50/1
  Delay48/1 -> Delay21/1
  [reord_dv] -> Gateway Out3/1
  [reord_sync] -> Gateway Out16/1
  Logical6/1 -> Delay24/1
  [fft_dvalid] -> Logical6/1
  Inverter/1 -> Logical6/2
  Mux1/1 -> [reord_pol0]
  Single Port RAM/1 -> Mux1/2
  Delay92/1 -> Delay45/1, AddSub/1
  [current_channel] -> Delay92/1
  Delay88/1 -> Delay93/1
  Delay93/1 -> Delay94/1
  Delay94/1 -> Mux1/3
  Delay113/1 -> Mux1/1, Delay114/1
  Delay4/1 -> Single Port RAM/3, Gateway Out47/1
  Slice4/1 -> Gateway Out55/1, Delay47/1
  Logical8/1 -> Register12/2, Gateway Out43/1, Delay55/1
  Register12/1 -> Gateway Out27/1, Logical8/2
  [fft_dvalid] -> Logical5/1, Delay95/1
  Delay50/1 -> Delay48/1
  Delay95/1 -> Gateway Out58/1, Delay50/1
  [data_pol1] -> Delay91/1, Delay101/1
  [current_channel] -> Slice6/1, Slice3/1
  Slice3/1 -> Delay115/1, Inverter3/1
  Delay65/1 -> Single Port RAM1/1
  Delay87/1 -> Delay90/1
  Delay91/1 -> Delay63/1
  Delay96/1 -> Delay65/1
  Logical10/1 -> Delay87/1
  [fft_dvalid] -> Logical10/1
  Inverter3/1 -> Logical10/2
  Single Port RAM1/1 -> Mux11/2
  Delay101/1 -> Delay103/1
  Delay103/1 -> Delay104/1
  Delay104/1 -> Mux11/3
  Delay117/1 -> Mux11/1
  Delay90/1 -> Single Port RAM1/3
  Slice6/1 -> Delay96/1
  Mux11/1 -> [reord_pol1]
  [reord_mux_sel_ext] -> pipeline43/1(d)
  pipeline43/1(q) -> ss_nb_sync/9(in_reord_mux_sel)
  [sync_out] -> [new_spec]
  pipeline45/1(q) -> Delay107/1
  pipeline2/1(q) -> Delay108/1
  Logical1/1 -> Fast Fourier Transform 9.0 1/6
  Gateway Out48/1 -> To Workspace53/1
  Gateway Out53/1 -> To Workspace54/1
  edge_detect9/1(out) -> Gateway Out48/1, [fir_data_tlast]
  Delay68/1 -> edge_detect9/1(in)
  Delay89/1 -> edge_detect10/1(in)
  Delay97/1 -> Logical11/2
  [fir_sync] -> Delay98/1, Logical7/1
  Delay98/1 -> Logical7/2
  [fir_sync] -> pipeline229/1(d)
  Delay21/1 -> [reord_dv]
  Delay99/1 -> [reord_channel]
  [reord_sync] -> Register6/3, Register6/1
  Register6/1 -> Logical3/1
  Logical3/1 -> Delay43/1, Register6/2
  Delay63/1 -> Single Port RAM1/2
  Gateway Out19/1 -> To Workspace18/1
  Gateway Out27/1 -> To Workspace31/1
  Gateway Out33/1 -> To Workspace34/1
  Gateway Out43/1 -> To Workspace43/1
  Gateway Out55/1 -> To Workspace56/1
  Logical5/1 -> Delay102/1
  Slice2/1 -> Delay111/1, [reord_mux_sel], Inverter/1
  [reord_mux_sel] -> Gateway Out56/1, Logical5/2
  Gateway Out56/1 -> To Workspace57/1
  Delay45/1 -> Delay86/1
  Delay86/1 -> Delay100/1
  Gateway Out57/1 -> To Workspace58/1
  Delay100/1 -> Gateway Out57/1, [reg_channel]
  Delay102/1 -> Gateway Out19/1, Logical8/1
  Gateway Out58/1 -> To Workspace59/1
  [capture_now] -> Logical3/2
  Delay106/1 -> [nb_dv]
  Delay107/1 -> [pol0]
  Delay108/1 -> [pol1]
  Delay49/1 -> Delay110/1
  edge_detect10/1(out) -> [fir_sync], Gateway Out6/1
  Fast Fourier Transform 9.0 1/9 -> pipeline124/1(d), Delay109/1
  [sync_out] -> Counter1/2
  [cnt_rst] -> Counter1/1
  Delay110/1 -> [reord_sync]
  Slice5/1 -> pipeline39/1(d)
  pipeline49/1(q) -> ss_nb/11(in_ch)
  Delay105/1 -> [fft_ch_out]
  [fft_ch_out] -> Gateway Out83/1
  [fft_ch_out] -> pipeline49/1(d)
  Delay111/1 -> Delay112/1
  Delay112/1 -> Delay113/1
  Delay114/1 -> [reord_mux_sel_ext]
  pipeline33/1(q) -> ss_nb_sync/5(in_re_ord_ch)
  pipeline51/1(q) -> ss_nb_sync/10(in_reg_ch)
  [reg_channel] -> pipeline51/1(d)
  Delay116/1 -> Delay117/1
  Delay115/1 -> Delay116/1
  Constant/1 -> Relational2/2
  Relational2/1 -> Logical/1
  Logical/1 -> edge_detect1/1(in)
  Delay109/1 -> Logical/2
  Delay118/1 -> Inverter4/1, Register5/1, Register5/3
  Inverter4/1 -> Logical/3
  Fast Fourier Transform 9.0 2/1 -> Terminator1/1
  Fast Fourier Transform 9.0 2/10 -> Terminator12/1
  Fast Fourier Transform 9.0 2/17 -> Terminator4/1
  Fast Fourier Transform 9.0 2/16 -> Terminator3/1
  Fast Fourier Transform 9.0 2/15 -> Terminator2/1
  Fast Fourier Transform 9.0 2/13 -> Terminator11/1
  Fast Fourier Transform 9.0 2/11 -> Terminator13/1
  Fast Fourier Transform 9.0 2/12 -> Terminator21/1
  Fast Fourier Transform 9.0 2/2 -> Terminator14/1
  Fast Fourier Transform 9.0 2/9 -> pipeline50/1(d)
  Fast Fourier Transform 9.0 2/8 -> pipeline12/1(d)
  Fast Fourier Transform 9.0 2/6 -> pipeline48/1(d)
  Fast Fourier Transform 9.0 2/5 -> pipeline44/1(d)
  Constant5/1 -> Fast Fourier Transform 9.0 2/2
  Fast Fourier Transform 9.0 2/3 -> Terminator15/1
  Fast Fourier Transform 9.0 2/4 -> Terminator16/1
  pipeline5/1(q) -> [fft_pol1_of]
  [fft_pol1_of] -> Concat2/2
  [fft_pol0_of] -> Concat2/1
  Concat2/1 -> pfb_of/1
  Constant4/1 -> Fast Fourier Transform 9.0 1/9
  Constant11/1 -> Fast Fourier Transform 9.0 2/8
  Fast Fourier Transform 9.0 1/3 -> Terminator17/1
  Fast Fourier Transform 9.0 1/4 -> Terminator18/1
  Fast Fourier Transform 9.0 1/13 -> Terminator20/1
  Fast Fourier Transform 9.0 1/12 -> Terminator22/1
  Fast Fourier Transform 9.0 1/11 -> Terminator23/1
  Fast Fourier Transform 9.0 1/10 -> Terminator24/1
  pipeline16/1(q) -> [fft_pol0_of]
  [fft_shift] -> register_change_detect/1(data)
  register_change_detect/1(state_change) -> edge_detect7/1(in)
  edge_detect7/1(out) -> [fft_config_reload]
  Fast Fourier Transform 9.0 1/7 -> Terminator19/1
  Fast Fourier Transform 9.0 1/14 -> pipeline16/1(d)
  Fast Fourier Transform 9.0 2/14 -> pipeline5/1(d)
  Fast Fourier Transform 9.0 2/7 -> Terminator10/1
  Counter2/1 -> fft_shift_change/1(out_reg)
  pipeline3/1(q) -> Counter2/1
  [cnt_rst] -> pipeline3/1(d)
  pipeline22/1(q) -> Counter2/2
  [fft_config_reload] -> pipeline22/1(d)
  Register/1 -> fft_shift_value/1(out_reg)
  [cnt_rst] -> Register/2
  pipeline23/1(q) -> [fft_conf_tready_p0]
  pipeline24/1(q) -> ss_fft/7(in_conf_trdy)
  [fft_conf_tready_p0] -> pipeline24/1(d)
  [fft_config_reload] -> Register/3
